simulink library "lib_LargeBuildingModel"  (R2026a)
settings: Solver=VariableStepAuto
libraries: WallSelector_lib x380, ExternalWall_lib x188, RoomWithAirVolume x140, fl_lib x139, RoomLevelControl_lib x1
(part 6 of 12)

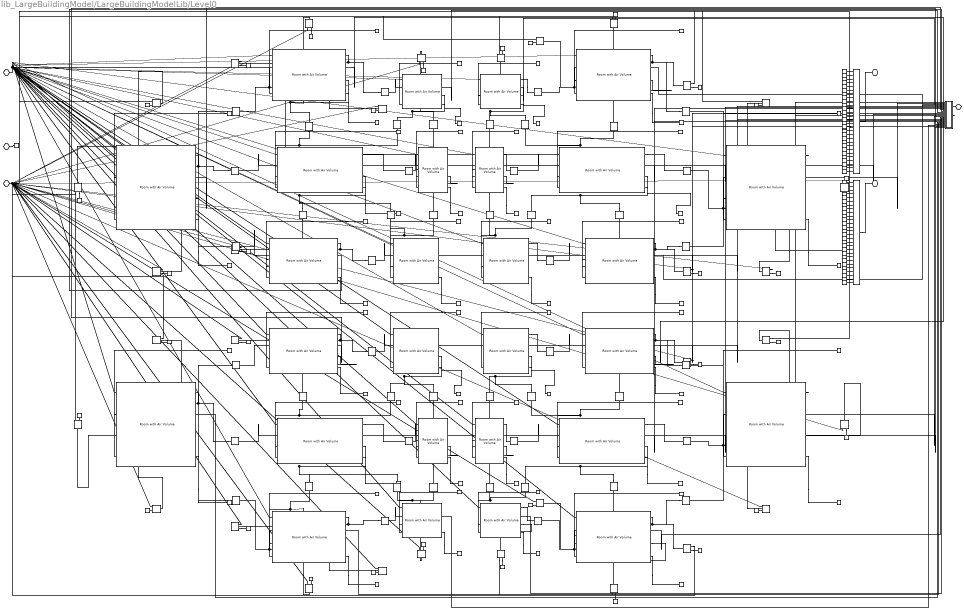
== system lib_LargeBuildingModel/LargeBuildingModelLib/Level0 ==
  note: A1R1 (LivingRoom_A)
  note: A1R2 (Bedroom_A)
  note: A1R3 (Kitchen_A)
  note: A1R4 (Bathroom_A)
  note: A1R5 (FireExit_A)
  note: A1R6 (Lobby1_A)
  note: A1R7 (Lobby2_A)
  note: A2R1 (LivingRoom_B)
  note: A2R2 (Bedroom_B)
  note: A2R3 (Kitchen_B)
  note: A2R4 (Bathroom_B)
  note: A2R5 (FireExit_B)
  note: A2R6 (Lobby1_B)
  note: A2R7 (Lobby2_B)
  note: A3R1 (LivingRoom_C)
  note: A3R2 (Bedroom_C)
  note: A3R3 (Kitchen_C)
  note: A3R4 (Bathroom_C)
  note: A3R5 (FireExit_C)
  note: A3R6 (Lobby1_C)
  note: A3R7 (Lobby2_C)
  note: A4R1 (LivingRoom_D)
  note: A4R2 (Bedroom_D)
  note: A4R3 (Kitchen_D)
  note: A4R4 (Bathroom_D)
  note: A4R5 (FireExit_D)
  note: A4R6 (Lobby1_D)
  note: A4R7 (Lobby2_D)
  Amb{1..32} (32 alike) : ConnectionLabel  Label=A
  AmbPort : ConnectionLabel  Label=A
  ArrayBottom : SimscapeArrayConnection  Domain=foundation.thermal.thermal  ConcatenateDimension=1  NumScalarElements=28
  ArrayTop : SimscapeArrayConnection  Domain=foundation.thermal.thermal  ConcatenateDimension=1  NumScalarElements=28
  Bottom1 : ConnectionLabel  Label=Bottom1
  Bottom10 : ConnectionLabel  Label=Bottom10
  Bottom10Lib : ConnectionLabel  Label=Bottom10
  Bottom11 : ConnectionLabel  Label=Bottom11
  Bottom11Lib : ConnectionLabel  Label=Bottom11
  Bottom12 : ConnectionLabel  Label=Bottom12
  Bottom12Lib : ConnectionLabel  Label=Bottom12
  Bottom13 : ConnectionLabel  Label=Bottom13
  Bottom13Lib : ConnectionLabel  Label=Bottom13
  Bottom14 : ConnectionLabel  Label=Bottom14
  Bottom14Lib : ConnectionLabel  Label=Bottom14
  Bottom15 : ConnectionLabel  Label=Bottom15
  Bottom15Lib : ConnectionLabel  Label=Bottom15
  Bottom16 : ConnectionLabel  Label=Bottom16
  Bottom16Lib : ConnectionLabel  Label=Bottom16
  Bottom17 : ConnectionLabel  Label=Bottom17
  Bottom17Lib : ConnectionLabel  Label=Bottom17
  Bottom18 : ConnectionLabel  Label=Bottom18
  Bottom18Lib : ConnectionLabel  Label=Bottom18
  Bottom19 : ConnectionLabel  Label=Bottom19
  Bottom19Lib : ConnectionLabel  Label=Bottom19
  Bottom1Lib : ConnectionLabel  Label=Bottom1
  Bottom2 : ConnectionLabel  Label=Bottom2
  Bottom20 : ConnectionLabel  Label=Bottom20
  Bottom20Lib : ConnectionLabel  Label=Bottom20
  Bottom21 : ConnectionLabel  Label=Bottom21
  Bottom21Lib : ConnectionLabel  Label=Bottom21
  Bottom22 : ConnectionLabel  Label=Bottom22
  Bottom22Lib : ConnectionLabel  Label=Bottom22
  Bottom23 : ConnectionLabel  Label=Bottom23
  Bottom23Lib : ConnectionLabel  Label=Bottom23
  Bottom24 : ConnectionLabel  Label=Bottom24
  Bottom24Lib : ConnectionLabel  Label=Bottom24
  Bottom25 : ConnectionLabel  Label=Bottom25
  Bottom25Lib : ConnectionLabel  Label=Bottom25
  Bottom26 : ConnectionLabel  Label=Bottom26
  Bottom26Lib : ConnectionLabel  Label=Bottom26
  Bottom27 : ConnectionLabel  Label=Bottom27
  Bottom27Lib : ConnectionLabel  Label=Bottom27
  Bottom28 : ConnectionLabel  Label=Bottom28
  Bottom28Lib : ConnectionLabel  Label=Bottom28
  Bottom2Lib : ConnectionLabel  Label=Bottom2
  Bottom3 : ConnectionLabel  Label=Bottom3
  Bottom3Lib : ConnectionLabel  Label=Bottom3
  Bottom4 : ConnectionLabel  Label=Bottom4
  Bottom4Lib : ConnectionLabel  Label=Bottom4
  Bottom5 : ConnectionLabel  Label=Bottom5
  Bottom5Lib : ConnectionLabel  Label=Bottom5
  Bottom6 : ConnectionLabel  Label=Bottom6
  Bottom6Lib : ConnectionLabel  Label=Bottom6
  Bottom7 : ConnectionLabel  Label=Bottom7
  Bottom7Lib : ConnectionLabel  Label=Bottom7
  Bottom8 : ConnectionLabel  Label=Bottom8
  Bottom8Lib : ConnectionLabel  Label=Bottom8
  Bottom9 : ConnectionLabel  Label=Bottom9
  Bottom9Lib : ConnectionLabel  Label=Bottom9
  ExtWall (A1R2W1) : ExternalWall_lib/Wall External  extWallModel=wallExternalModelOption.wallSolarWin  wallLength=4.2672 % Parameterized on : 13-Jun-2026 10:47:11 m  wallHeight=3.048 % Parameterized on : 13-Jun-2026 10:47:11 m  wallThickness=0.07 % Parameterized on : 13-Jun-2026 10:47:11 m  wallMaterialDen=2000 % Parameterized on : 13-Jun-2026 10:47:16 kg/m^3  wallMaterialCp=1100 % Parameterized on : 13-Jun-2026 10:47:16 J/(K*kg)  wallAbsorptivity=0.6 % Parameterized on : 13-Jun-2026 10:47:16  wallThermalK=1.4 % Parameterized on : 13-Jun-2026 10:47:16 W/(K*m)  winLength=3.0174 % Parameterized on : 13-Jun-2026 10:47:11 m  winHeight=2.1553 % Parameterized on : 13-Jun-2026 10:47:11 m  winThickness=0.005 % Parameterized on : 13-Jun-2026 10:47:16 m  winMaterialDen=4000 % Parameterized on : 13-Jun-2026 10:47:17 kg/m^3  winMaterialCp=840 % Parameterized on : 13-Jun-2026 10:47:17 J/(K*kg)  winAbsorptivity=0.4 % Parameterized on : 13-Jun-2026 10:47:17  winThermalK=1 % Parameterized on : 13-Jun-2026 10:47:17 W/(K*m)  winTransmissivity=0.2 % Parameterized on : 13-Jun-2026 10:47:17  ventLength=0.1 m  ventHeight=0.1 m  extToWallHTC=20 % Parameterized on : 13-Jun-2026 10:47:16 W/(K*m^2)  intToRoomHTC=30 % Parameterized on : 13-Jun-2026 10:47:16 W/(K*m^2)  iniT=300 % Parameterized on : 13-Jun-2026 10:47:16 K  latitude=5  longitude=5  localTime=5  dayLightS=0  surfAngle=90 % Parameterized on : 13-Jun-2026 10:47:11 deg  surfUnitV=[0 -1] % Parameterized on : 13-Jun-2026 10:47:11  startYear=2025  startMonth=1  startDay=1  startHr=1  numHrsData=24  interp_method=simscape.enum.interpolation.linear  extrap_method=simscape.enum.extrapolation.nearest
  ExtWall (A1R2W3) : ExternalWall_lib/Wall External  extWallModel=wallExternalModelOption.wallSolarWin  wallLength=4.2672 % Parameterized on : 13-Jun-2026 10:47:11 m  wallHeight=3.048 % Parameterized on : 13-Jun-2026 10:47:11 m  wallThickness=0.07 % Parameterized on : 13-Jun-2026 10:47:11 m  wallMaterialDen=2000 % Parameterized on : 13-Jun-2026 10:47:17 kg/m^3  wallMaterialCp=1100 % Parameterized on : 13-Jun-2026 10:47:17 J/(K*kg)  wallAbsorptivity=0.6 % Parameterized on : 13-Jun-2026 10:47:17  wallThermalK=1.4 % Parameterized on : 13-Jun-2026 10:47:17 W/(K*m)  winLength=3.3054 % Parameterized on : 13-Jun-2026 10:47:12 m  winHeight=2.361 % Parameterized on : 13-Jun-2026 10:47:12 m  winThickness=0.005 % Parameterized on : 13-Jun-2026 10:47:17 m  winMaterialDen=4000 % Parameterized on : 13-Jun-2026 10:47:17 kg/m^3  winMaterialCp=840 % Parameterized on : 13-Jun-2026 10:47:17 J/(K*kg)  winAbsorptivity=0.4 % Parameterized on : 13-Jun-2026 10:47:17  winThermalK=1 % Parameterized on : 13-Jun-2026 10:47:17 W/(K*m)  winTransmissivity=0.2 % Parameterized on : 13-Jun-2026 10:47:17  ventLength=0.1 m  ventHeight=0.1 m  extToWallHTC=20 % Parameterized on : 13-Jun-2026 10:47:17 W/(K*m^2)  intToRoomHTC=30 % Parameterized on : 13-Jun-2026 10:47:17 W/(K*m^2)  iniT=300 % Parameterized on : 13-Jun-2026 10:47:17 K  latitude=5  longitude=5  localTime=5  dayLightS=0  surfAngle=90 % Parameterized on : 13-Jun-2026 10:47:11 deg  surfUnitV="[0  1] % Parameterized on : 13-Jun-2026 10:47:11"  startYear=2025  startMonth=1  startDay=1  startHr=1  numHrsData=24  interp_method=simscape.enum.interpolation.linear  extrap_method=simscape.enum.extrapolation.nearest
  ExtWall (A1R2W4) : ExternalWall_lib/Wall External  extWallModel=wallExternalModelOption.wallSolar  wallLength=4.572 % Parameterized on : 13-Jun-2026 10:47:12 m  wallHeight=3.048 % Parameterized on : 13-Jun-2026 10:47:12 m  wallThickness=0.07 % Parameterized on : 13-Jun-2026 10:47:12 m  wallMaterialDen=2000 % Parameterized on : 13-Jun-2026 10:47:17 kg/m^3  wallMaterialCp=1100 % Parameterized on : 13-Jun-2026 10:47:17 J/(K*kg)  wallAbsorptivity=0.6 % Parameterized on : 13-Jun-2026 10:47:17  wallThermalK=1.4 % Parameterized on : 13-Jun-2026 10:47:17 W/(K*m)  winLength=1 m  winHeight=0.5 m  winThickness=0.007 m  winMaterialDen=2500 kg/m^3  winMaterialCp=787 J/(K*kg)  winAbsorptivity=0.35  winThermalK=1 W/(K*m)  winTransmissivity=0.45  ventLength=0.1 m  ventHeight=0.1 m  extToWallHTC=20 % Parameterized on : 13-Jun-2026 10:47:17 W/(K*m^2)  intToRoomHTC=30 % Parameterized on : 13-Jun-2026 10:47:17 W/(K*m^2)  iniT=300 % Parameterized on : 13-Jun-2026 10:47:17 K  latitude=5  longitude=5  localTime=5  dayLightS=0  surfAngle=90 % Parameterized on : 13-Jun-2026 10:47:12 deg  surfUnitV="[1  0] % Parameterized on : 13-Jun-2026 10:47:12"  startYear=2025  startMonth=1  startDay=1  startHr=1  numHrsData=24  interp_method=simscape.enum.interpolation.linear  extrap_method=simscape.enum.extrapolation.nearest
  ExtWall (A1R3W1) : ExternalWall_lib/Wall External  extWallModel=wallExternalModelOption.wallSolarWin  wallLength=2.7432 % Parameterized on : 13-Jun-2026 10:47:12 m  wallHeight=3.048 % Parameterized on : 13-Jun-2026 10:47:12 m  wallThickness=0.07 % Parameterized on : 13-Jun-2026 10:47:12 m  wallMaterialDen=2000 % Parameterized on : 13-Jun-2026 10:47:17 kg/m^3  wallMaterialCp=1100 % Parameterized on : 13-Jun-2026 10:47:17 J/(K*kg)  wallAbsorptivity=0.6 % Parameterized on : 13-Jun-2026 10:47:17  wallThermalK=1.4 % Parameterized on : 13-Jun-2026 10:47:17 W/(K*m)  winLength=2.4536 % Parameterized on : 13-Jun-2026 10:47:12 m  winHeight=2.7262 % Parameterized on : 13-Jun-2026 10:47:12 m  winThickness=0.005 % Parameterized on : 13-Jun-2026 10:47:17 m  winMaterialDen=4000 % Parameterized on : 13-Jun-2026 10:47:17 kg/m^3  winMaterialCp=840 % Parameterized on : 13-Jun-2026 10:47:17 J/(K*kg)  winAbsorptivity=0.4 % Parameterized on : 13-Jun-2026 10:47:17  winThermalK=1 % Parameterized on : 13-Jun-2026 10:47:17 W/(K*m)  winTransmissivity=0.2 % Parameterized on : 13-Jun-2026 10:47:17  ventLength=0.1 m  ventHeight=0.1 m  extToWallHTC=20 % Parameterized on : 13-Jun-2026 10:47:17 W/(K*m^2)  intToRoomHTC=30 % Parameterized on : 13-Jun-2026 10:47:17 W/(K*m^2)  iniT=300 % Parameterized on : 13-Jun-2026 10:47:17 K  latitude=5  longitude=5  localTime=5  dayLightS=0  surfAngle=90 % Parameterized on : 13-Jun-2026 10:47:12 deg  surfUnitV="[-1  0] % Parameterized on : 13-Jun-2026 10:47:12"  startYear=2025  startMonth=1  startDay=1  startHr=1  numHrsData=24  interp_method=simscape.enum.interpolation.linear  extrap_method=simscape.enum.extrapolation.nearest
  ExtWall (A1R3W3) : ExternalWall_lib/Wall External  extWallModel=wallExternalModelOption.wallSolarWin  wallLength=2.7432 % Parameterized on : 13-Jun-2026 10:47:12 m  wallHeight=3.048 % Parameterized on : 13-Jun-2026 10:47:12 m  wallThickness=0.07 % Parameterized on : 13-Jun-2026 10:47:12 m  wallMaterialDen=2000 % Parameterized on : 13-Jun-2026 10:47:17 kg/m^3  wallMaterialCp=1100 % Parameterized on : 13-Jun-2026 10:47:17 J/(K*kg)  wallAbsorptivity=0.6 % Parameterized on : 13-Jun-2026 10:47:17  wallThermalK=1.4 % Parameterized on : 13-Jun-2026 10:47:17 W/(K*m)  winLength=1.9397 % Parameterized on : 13-Jun-2026 10:47:12 m  winHeight=2.1553 % Parameterized on : 13-Jun-2026 10:47:12 m  winThickness=0.005 % Parameterized on : 13-Jun-2026 10:47:17 m  winMaterialDen=4000 % Parameterized on : 13-Jun-2026 10:47:17 kg/m^3  winMaterialCp=840 % Parameterized on : 13-Jun-2026 10:47:17 J/(K*kg)  winAbsorptivity=0.4 % Parameterized on : 13-Jun-2026 10:47:17  winThermalK=1 % Parameterized on : 13-Jun-2026 10:47:17 W/(K*m)  winTransmissivity=0.2 % Parameterized on : 13-Jun-2026 10:47:17  ventLength=0.1 m  ventHeight=0.1 m  extToWallHTC=20 % Parameterized on : 13-Jun-2026 10:47:17 W/(K*m^2)  intToRoomHTC=30 % Parameterized on : 13-Jun-2026 10:47:17 W/(K*m^2)  iniT=300 % Parameterized on : 13-Jun-2026 10:47:17 K  latitude=5  longitude=5  localTime=5  dayLightS=0  surfAngle=90 % Parameterized on : 13-Jun-2026 10:47:12 deg  surfUnitV="[1  0] % Parameterized on : 13-Jun-2026 10:47:12"  startYear=2025  startMonth=1  startDay=1  startHr=1  numHrsData=24  interp_method=simscape.enum.interpolation.linear  extrap_method=simscape.enum.extrapolation.nearest
  ExtWall (A1R3W4) : ExternalWall_lib/Wall External  extWallModel=wallExternalModelOption.wallSolar  wallLength=3.9624 % Parameterized on : 13-Jun-2026 10:47:12 m  wallHeight=3.048 % Parameterized on : 13-Jun-2026 10:47:12 m  wallThickness=0.07 % Parameterized on : 13-Jun-2026 10:47:12 m  wallMaterialDen=2000 % Parameterized on : 13-Jun-2026 10:47:17 kg/m^3  wallMaterialCp=1100 % Parameterized on : 13-Jun-2026 10:47:17 J/(K*kg)  wallAbsorptivity=0.6 % Parameterized on : 13-Jun-2026 10:47:17  wallThermalK=1.4 % Parameterized on : 13-Jun-2026 10:47:17 W/(K*m)  winLength=1 m  winHeight=0.5 m  winThickness=0.007 m  winMaterialDen=2500 kg/m^3  winMaterialCp=787 J/(K*kg)  winAbsorptivity=0.35  winThermalK=1 W/(K*m)  winTransmissivity=0.45  ventLength=0.1 m  ventHeight=0.1 m  extToWallHTC=20 % Parameterized on : 13-Jun-2026 10:47:17 W/(K*m^2)  intToRoomHTC=30 % Parameterized on : 13-Jun-2026 10:47:17 W/(K*m^2)  iniT=300 % Parameterized on : 13-Jun-2026 10:47:17 K  latitude=5  longitude=5  localTime=5  dayLightS=0  surfAngle=90 % Parameterized on : 13-Jun-2026 10:47:12 deg  surfUnitV=[0 -1] % Parameterized on : 13-Jun-2026 10:47:12  startYear=2025  startMonth=1  startDay=1  startHr=1  numHrsData=24  interp_method=simscape.enum.interpolation.linear  extrap_method=simscape.enum.extrapolation.nearest
  ExtWall (A1R4W3) : ExternalWall_lib/Wall External  extWallModel=wallExternalModelOption.wallSolar  wallLength=2.4384 % Parameterized on : 13-Jun-2026 10:47:12 m  wallHeight=3.048 % Parameterized on : 13-Jun-2026 10:47:12 m  wallThickness=0.07 % Parameterized on : 13-Jun-2026 10:47:12 m  wallMaterialDen=2000 % Parameterized on : 13-Jun-2026 10:47:17 kg/m^3  wallMaterialCp=1100 % Parameterized on : 13-Jun-2026 10:47:17 J/(K*kg)  wallAbsorptivity=0.6 % Parameterized on : 13-Jun-2026 10:47:17  wallThermalK=1.4 % Parameterized on : 13-Jun-2026 10:47:17 W/(K*m)  winLength=1 m  winHeight=0.5 m  winThickness=0.007 m  winMaterialDen=2500 kg/m^3  winMaterialCp=787 J/(K*kg)  winAbsorptivity=0.35  winThermalK=1 W/(K*m)  winTransmissivity=0.45  ventLength=0.1 m  ventHeight=0.1 m  extToWallHTC=20 % Parameterized on : 13-Jun-2026 10:47:17 W/(K*m^2)  intToRoomHTC=30 % Parameterized on : 13-Jun-2026 10:47:17 W/(K*m^2)  iniT=300 % Parameterized on : 13-Jun-2026 10:47:17 K  latitude=5  longitude=5  localTime=5  dayLightS=0  surfAngle=90 % Parameterized on : 13-Jun-2026 10:47:12 deg  surfUnitV="[1  0] % Parameterized on : 13-Jun-2026 10:47:12"  startYear=2025  startMonth=1  startDay=1  startHr=1  numHrsData=24  interp_method=simscape.enum.interpolation.linear  extrap_method=simscape.enum.extrapolation.nearest
  ExtWall (A1R5W4) : ExternalWall_lib/Wall External  extWallModel=wallExternalModelOption.wallSolar  wallLength=2.1336 % Parameterized on : 13-Jun-2026 10:47:12 m  wallHeight=3.048 % Parameterized on : 13-Jun-2026 10:47:12 m  wallThickness=0.07 % Parameterized on : 13-Jun-2026 10:47:12 m  wallMaterialDen=2000 % Parameterized on : 13-Jun-2026 10:47:17 kg/m^3  wallMaterialCp=1100 % Parameterized on : 13-Jun-2026 10:47:17 J/(K*kg)  wallAbsorptivity=0.6 % Parameterized on : 13-Jun-2026 10:47:17  wallThermalK=1.4 % Parameterized on : 13-Jun-2026 10:47:17 W/(K*m)  winLength=1 m  winHeight=0.5 m  winThickness=0.007 m  winMaterialDen=2500 kg/m^3  winMaterialCp=787 J/(K*kg)  winAbsorptivity=0.35  winThermalK=1 W/(K*m)  winTransmissivity=0.45  ventLength=0.1 m  ventHeight=0.1 m  extToWallHTC=20 % Parameterized on : 13-Jun-2026 10:47:17 W/(K*m^2)  intToRoomHTC=30 % Parameterized on : 13-Jun-2026 10:47:17 W/(K*m^2)  iniT=300 % Parameterized on : 13-Jun-2026 10:47:17 K  latitude=5  longitude=5  localTime=5  dayLightS=0  surfAngle=90 % Parameterized on : 13-Jun-2026 10:47:12 deg  surfUnitV="[-6.0708e-17          -1] % Parameterized on : 13-Jun-2026 10:47:12"  startYear=2025  startMonth=1  startDay=1  startHr=1  numHrsData=24  interp_method=simscape.enum.interpolation.linear  extrap_method=simscape.enum.extrapolation.nearest
  ExtWall (A2R2W1) : ExternalWall_lib/Wall External  extWallModel=wallExternalModelOption.wallSolarWin  wallLength=4.2672 % Parameterized on : 13-Jun-2026 10:47:12 m  wallHeight=3.048 % Parameterized on : 13-Jun-2026 10:47:12 m  wallThickness=0.07 % Parameterized on : 13-Jun-2026 10:47:12 m  wallMaterialDen=2000 % Parameterized on : 13-Jun-2026 10:47:17 kg/m^3  wallMaterialCp=1100 % Parameterized on : 13-Jun-2026 10:47:17 J/(K*kg)  wallAbsorptivity=0.6 % Parameterized on : 13-Jun-2026 10:47:17  wallThermalK=1.4 % Parameterized on : 13-Jun-2026 10:47:17 W/(K*m)  winLength=3.3054 % Parameterized on : 13-Jun-2026 10:47:12 m  winHeight=2.361 % Parameterized on : 13-Jun-2026 10:47:12 m  winThickness=0.005 % Parameterized on : 13-Jun-2026 10:47:17 m  winMaterialDen=4000 % Parameterized on : 13-Jun-2026 10:47:17 kg/m^3  winMaterialCp=840 % Parameterized on : 13-Jun-2026 10:47:17 J/(K*kg)  winAbsorptivity=0.4 % Parameterized on : 13-Jun-2026 10:47:17  winThermalK=1 % Parameterized on : 13-Jun-2026 10:47:17 W/(K*m)  winTransmissivity=0.2 % Parameterized on : 13-Jun-2026 10:47:17  ventLength=0.1 m  ventHeight=0.1 m  extToWallHTC=20 % Parameterized on : 13-Jun-2026 10:47:17 W/(K*m^2)  intToRoomHTC=30 % Parameterized on : 13-Jun-2026 10:47:17 W/(K*m^2)  iniT=300 % Parameterized on : 13-Jun-2026 10:47:17 K  latitude=5  longitude=5  localTime=5  dayLightS=0  surfAngle=90 % Parameterized on : 13-Jun-2026 10:47:12 deg  surfUnitV=[0 -1] % Parameterized on : 13-Jun-2026 10:47:12  startYear=2025  startMonth=1  startDay=1  startHr=1  numHrsData=24  interp_method=simscape.enum.interpolation.linear  extrap_method=simscape.enum.extrapolation.nearest
  ExtWall (A2R2W2) : ExternalWall_lib/Wall External  extWallModel=wallExternalModelOption.wallSolar  wallLength=4.572 % Parameterized on : 13-Jun-2026 10:47:12 m  wallHeight=3.048 % Parameterized on : 13-Jun-2026 10:47:12 m  wallThickness=0.07 % Parameterized on : 13-Jun-2026 10:47:12 m  wallMaterialDen=2000 % Parameterized on : 13-Jun-2026 10:47:17 kg/m^3  wallMaterialCp=1100 % Parameterized on : 13-Jun-2026 10:47:17 J/(K*kg)  wallAbsorptivity=0.6 % Parameterized on : 13-Jun-2026 10:47:17  wallThermalK=1.4 % Parameterized on : 13-Jun-2026 10:47:17 W/(K*m)  winLength=1 m  winHeight=0.5 m  winThickness=0.007 m  winMaterialDen=2500 kg/m^3  winMaterialCp=787 J/(K*kg)  winAbsorptivity=0.35  winThermalK=1 W/(K*m)  winTransmissivity=0.45  ventLength=0.1 m  ventHeight=0.1 m  extToWallHTC=20 % Parameterized on : 13-Jun-2026 10:47:17 W/(K*m^2)  intToRoomHTC=30 % Parameterized on : 13-Jun-2026 10:47:17 W/(K*m^2)  iniT=300 % Parameterized on : 13-Jun-2026 10:47:17 K  latitude=5  longitude=5  localTime=5  dayLightS=0  surfAngle=90 % Parameterized on : 13-Jun-2026 10:47:12 deg  surfUnitV="[-1  0] % Parameterized on : 13-Jun-2026 10:47:12"  startYear=2025  startMonth=1  startDay=1  startHr=1  numHrsData=24  interp_method=simscape.enum.interpolation.linear  extrap_method=simscape.enum.extrapolation.nearest
  ExtWall (A2R2W3) : ExternalWall_lib/Wall External  extWallModel=wallExternalModelOption.wallSolarWin  wallLength=4.2672 % Parameterized on : 13-Jun-2026 10:47:12 m  wallHeight=3.048 % Parameterized on : 13-Jun-2026 10:47:12 m  wallThickness=0.07 % Parameterized on : 13-Jun-2026 10:47:12 m  wallMaterialDen=2000 % Parameterized on : 13-Jun-2026 10:47:17 kg/m^3  wallMaterialCp=1100 % Parameterized on : 13-Jun-2026 10:47:17 J/(K*kg)  wallAbsorptivity=0.6 % Parameterized on : 13-Jun-2026 10:47:17  wallThermalK=1.4 % Parameterized on : 13-Jun-2026 10:47:17 W/(K*m)  winLength=3.8167 % Parameterized on : 13-Jun-2026 10:47:12 m  winHeight=2.7262 % Parameterized on : 13-Jun-2026 10:47:12 m  winThickness=0.005 % Parameterized on : 13-Jun-2026 10:47:17 m  winMaterialDen=4000 % Parameterized on : 13-Jun-2026 10:47:17 kg/m^3  winMaterialCp=840 % Parameterized on : 13-Jun-2026 10:47:17 J/(K*kg)  winAbsorptivity=0.4 % Parameterized on : 13-Jun-2026 10:47:17  winThermalK=1 % Parameterized on : 13-Jun-2026 10:47:17 W/(K*m)  winTransmissivity=0.2 % Parameterized on : 13-Jun-2026 10:47:17  ventLength=0.1 m  ventHeight=0.1 m  extToWallHTC=20 % Parameterized on : 13-Jun-2026 10:47:17 W/(K*m^2)  intToRoomHTC=30 % Parameterized on : 13-Jun-2026 10:47:17 W/(K*m^2)  iniT=300 % Parameterized on : 13-Jun-2026 10:47:17 K  latitude=5  longitude=5  localTime=5  dayLightS=0  surfAngle=90 % Parameterized on : 13-Jun-2026 10:47:12 deg  surfUnitV="[0  1] % Parameterized on : 13-Jun-2026 10:47:12"  startYear=2025  startMonth=1  startDay=1  startHr=1  numHrsData=24  interp_method=simscape.enum.interpolation.linear  extrap_method=simscape.enum.extrapolation.nearest
  ExtWall (A2R3W1) : ExternalWall_lib/Wall External  extWallModel=wallExternalModelOption.wallSolarWin  wallLength=2.7432 % Parameterized on : 13-Jun-2026 10:47:12 m  wallHeight=3.048 % Parameterized on : 13-Jun-2026 10:47:12 m  wallThickness=0.07 % Parameterized on : 13-Jun-2026 10:47:12 m  wallMaterialDen=2000 % Parameterized on : 13-Jun-2026 10:47:17 kg/m^3  wallMaterialCp=1100 % Parameterized on : 13-Jun-2026 10:47:17 J/(K*kg)  wallAbsorptivity=0.6 % Parameterized on : 13-Jun-2026 10:47:17  wallThermalK=1.4 % Parameterized on : 13-Jun-2026 10:47:17 W/(K*m)  winLength=1.9397 % Parameterized on : 13-Jun-2026 10:47:12 m  winHeight=2.1553 % Parameterized on : 13-Jun-2026 10:47:12 m  winThickness=0.005 % Parameterized on : 13-Jun-2026 10:47:17 m  winMaterialDen=4000 % Parameterized on : 13-Jun-2026 10:47:17 kg/m^3  winMaterialCp=840 % Parameterized on : 13-Jun-2026 10:47:17 J/(K*kg)  winAbsorptivity=0.4 % Parameterized on : 13-Jun-2026 10:47:17  winThermalK=1 % Parameterized on : 13-Jun-2026 10:47:17 W/(K*m)  winTransmissivity=0.2 % Parameterized on : 13-Jun-2026 10:47:17  ventLength=0.1 m  ventHeight=0.1 m  extToWallHTC=20 % Parameterized on : 13-Jun-2026 10:47:17 W/(K*m^2)  intToRoomHTC=30 % Parameterized on : 13-Jun-2026 10:47:17 W/(K*m^2)  iniT=300 % Parameterized on : 13-Jun-2026 10:47:17 K  latitude=5  longitude=5  localTime=5  dayLightS=0  surfAngle=90 % Parameterized on : 13-Jun-2026 10:47:12 deg  surfUnitV="[1  0] % Parameterized on : 13-Jun-2026 10:47:12"  startYear=2025  startMonth=1  startDay=1  startHr=1  numHrsData=24  interp_method=simscape.enum.interpolation.linear  extrap_method=simscape.enum.extrapolation.nearest
  ExtWall (A2R3W2) : ExternalWall_lib/Wall External  extWallModel=wallExternalModelOption.wallSolarWin  wallLength=3.9624 % Parameterized on : 13-Jun-2026 10:47:12 m  wallHeight=3.048 % Parameterized on : 13-Jun-2026 10:47:12 m  wallThickness=0.07 % Parameterized on : 13-Jun-2026 10:47:12 m  wallMaterialDen=2000 % Parameterized on : 13-Jun-2026 10:47:17 kg/m^3  wallMaterialCp=1100 % Parameterized on : 13-Jun-2026 10:47:17 J/(K*kg)  wallAbsorptivity=0.6 % Parameterized on : 13-Jun-2026 10:47:17  wallThermalK=1.4 % Parameterized on : 13-Jun-2026 10:47:17 W/(K*m)  winLength=2.8018 % Parameterized on : 13-Jun-2026 10:47:12 m  winHeight=2.1553 % Parameterized on : 13-Jun-2026 10:47:12 m  winThickness=0.005 % Parameterized on : 13-Jun-2026 10:47:17 m  winMaterialDen=4000 % Parameterized on : 13-Jun-2026 10:47:17 kg/m^3  winMaterialCp=840 % Parameterized on : 13-Jun-2026 10:47:17 J/(K*kg)  winAbsorptivity=0.4 % Parameterized on : 13-Jun-2026 10:47:17  winThermalK=1 % Parameterized on : 13-Jun-2026 10:47:17 W/(K*m)  winTransmissivity=0.2 % Parameterized on : 13-Jun-2026 10:47:17  ventLength=0.1 m  ventHeight=0.1 m  extToWallHTC=20 % Parameterized on : 13-Jun-2026 10:47:17 W/(K*m^2)  intToRoomHTC=30 % Parameterized on : 13-Jun-2026 10:47:17 W/(K*m^2)  iniT=300 % Parameterized on : 13-Jun-2026 10:47:17 K  latitude=5  longitude=5  localTime=5  dayLightS=0  surfAngle=90 % Parameterized on : 13-Jun-2026 10:47:12 deg  surfUnitV=[0 -1] % Parameterized on : 13-Jun-2026 10:47:12  startYear=2025  startMonth=1  startDay=1  startHr=1  numHrsData=24  interp_method=simscape.enum.interpolation.linear  extrap_method=simscape.enum.extrapolation.nearest
  ExtWall (A2R3W3) : ExternalWall_lib/Wall External  extWallModel=wallExternalModelOption.wallSolar  wallLength=2.7432 % Parameterized on : 13-Jun-2026 10:47:12 m  wallHeight=3.048 % Parameterized on : 13-Jun-2026 10:47:12 m  wallThickness=0.07 % Parameterized on : 13-Jun-2026 10:47:12 m  wallMaterialDen=2000 % Parameterized on : 13-Jun-2026 10:47:17 kg/m^3  wallMaterialCp=1100 % Parameterized on : 13-Jun-2026 10:47:17 J/(K*kg)  wallAbsorptivity=0.6 % Parameterized on : 13-Jun-2026 10:47:17  wallThermalK=1.4 % Parameterized on : 13-Jun-2026 10:47:17 W/(K*m)  winLength=1 m  winHeight=0.5 m  winThickness=0.007 m  winMaterialDen=2500 kg/m^3  winMaterialCp=787 J/(K*kg)  winAbsorptivity=0.35  winThermalK=1 W/(K*m)  winTransmissivity=0.45  ventLength=0.1 m  ventHeight=0.1 m  extToWallHTC=20 % Parameterized on : 13-Jun-2026 10:47:17 W/(K*m^2)  intToRoomHTC=30 % Parameterized on : 13-Jun-2026 10:47:17 W/(K*m^2)  iniT=300 % Parameterized on : 13-Jun-2026 10:47:17 K  latitude=5  longitude=5  localTime=5  dayLightS=0  surfAngle=90 % Parameterized on : 13-Jun-2026 10:47:12 deg  surfUnitV="[-1  0] % Parameterized on : 13-Jun-2026 10:47:12"  startYear=2025  startMonth=1  startDay=1  startHr=1  numHrsData=24  interp_method=simscape.enum.interpolation.linear  extrap_method=simscape.enum.extrapolation.nearest
  ExtWall (A2R4W3) : ExternalWall_lib/Wall External  extWallModel=wallExternalModelOption.wallSolar  wallLength=2.4384 % Parameterized on : 13-Jun-2026 10:47:12 m  wallHeight=3.048 % Parameterized on : 13-Jun-2026 10:47:12 m  wallThickness=0.07 % Parameterized on : 13-Jun-2026 10:47:12 m  wallMaterialDen=2000 % Parameterized on : 13-Jun-2026 10:47:17 kg/m^3  wallMaterialCp=1100 % Parameterized on : 13-Jun-2026 10:47:17 J/(K*kg)  wallAbsorptivity=0.6 % Parameterized on : 13-Jun-2026 10:47:17  wallThermalK=1.4 % Parameterized on : 13-Jun-2026 10:47:17 W/(K*m)  winLength=1 m  winHeight=0.5 m  winThickness=0.007 m  winMaterialDen=2500 kg/m^3  winMaterialCp=787 J/(K*kg)  winAbsorptivity=0.35  winThermalK=1 W/(K*m)  winTransmissivity=0.45  ventLength=0.1 m  ventHeight=0.1 m  extToWallHTC=20 % Parameterized on : 13-Jun-2026 10:47:17 W/(K*m^2)  intToRoomHTC=30 % Parameterized on : 13-Jun-2026 10:47:17 W/(K*m^2)  iniT=300 % Parameterized on : 13-Jun-2026 10:47:17 K  latitude=5  longitude=5  localTime=5  dayLightS=0  surfAngle=90 % Parameterized on : 13-Jun-2026 10:47:12 deg  surfUnitV="[-1  0] % Parameterized on : 13-Jun-2026 10:47:12"  startYear=2025  startMonth=1  startDay=1  startHr=1  numHrsData=24  interp_method=simscape.enum.interpolation.linear  extrap_method=simscape.enum.extrapolation.nearest
  ExtWall (A2R5W2) : ExternalWall_lib/Wall External  extWallModel=wallExternalModelOption.wallSolar  wallLength=2.1336 % Parameterized on : 13-Jun-2026 10:47:12 m  wallHeight=3.048 % Parameterized on : 13-Jun-2026 10:47:12 m  wallThickness=0.07 % Parameterized on : 13-Jun-2026 10:47:12 m  wallMaterialDen=2000 % Parameterized on : 13-Jun-2026 10:47:17 kg/m^3  wallMaterialCp=1100 % Parameterized on : 13-Jun-2026 10:47:17 J/(K*kg)  wallAbsorptivity=0.6 % Parameterized on : 13-Jun-2026 10:47:17  wallThermalK=1.4 % Parameterized on : 13-Jun-2026 10:47:17 W/(K*m)  winLength=1 m  winHeight=0.5 m  winThickness=0.007 m  winMaterialDen=2500 kg/m^3  winMaterialCp=787 J/(K*kg)  winAbsorptivity=0.35  winThermalK=1 W/(K*m)  winTransmissivity=0.45  ventLength=0.1 m  ventHeight=0.1 m  extToWallHTC=20 % Parameterized on : 13-Jun-2026 10:47:17 W/(K*m^2)  intToRoomHTC=30 % Parameterized on : 13-Jun-2026 10:47:17 W/(K*m^2)  iniT=300 % Parameterized on : 13-Jun-2026 10:47:17 K  latitude=5  longitude=5  localTime=5  dayLightS=0  surfAngle=90 % Parameterized on : 13-Jun-2026 10:47:12 deg  surfUnitV=[0 -1] % Parameterized on : 13-Jun-2026 10:47:12  startYear=2025  startMonth=1  startDay=1  startHr=1  numHrsData=24  interp_method=simscape.enum.interpolation.linear  extrap_method=simscape.enum.extrapolation.nearest
  ExtWall (A3R2W1) : ExternalWall_lib/Wall External  extWallModel=wallExternalModelOption.wallSolarWin  wallLength=4.2672 % Parameterized on : 13-Jun-2026 10:47:12 m  wallHeight=3.048 % Parameterized on : 13-Jun-2026 10:47:12 m  wallThickness=0.07 % Parameterized on : 13-Jun-2026 10:47:12 m  wallMaterialDen=2000 % Parameterized on : 13-Jun-2026 10:47:17 kg/m^3  wallMaterialCp=1100 % Parameterized on : 13-Jun-2026 10:47:17 J/(K*kg)  wallAbsorptivity=0.6 % Parameterized on : 13-Jun-2026 10:47:17  wallThermalK=1.4 % Parameterized on : 13-Jun-2026 10:47:17 W/(K*m)  winLength=3.3054 % Parameterized on : 13-Jun-2026 10:47:12 m  winHeight=2.361 % Parameterized on : 13-Jun-2026 10:47:12 m  winThickness=0.005 % Parameterized on : 13-Jun-2026 10:47:17 m  winMaterialDen=4000 % Parameterized on : 13-Jun-2026 10:47:17 kg/m^3  winMaterialCp=840 % Parameterized on : 13-Jun-2026 10:47:17 J/(K*kg)  winAbsorptivity=0.4 % Parameterized on : 13-Jun-2026 10:47:17  winThermalK=1 % Parameterized on : 13-Jun-2026 10:47:17 W/(K*m)  winTransmissivity=0.2 % Parameterized on : 13-Jun-2026 10:47:17  ventLength=0.1 m  ventHeight=0.1 m  extToWallHTC=20 % Parameterized on : 13-Jun-2026 10:47:17 W/(K*m^2)  intToRoomHTC=30 % Parameterized on : 13-Jun-2026 10:47:17 W/(K*m^2)  iniT=300 % Parameterized on : 13-Jun-2026 10:47:17 K  latitude=5  longitude=5  localTime=5  dayLightS=0  surfAngle=90 % Parameterized on : 13-Jun-2026 10:47:12 deg  surfUnitV="[0  1] % Parameterized on : 13-Jun-2026 10:47:12"  startYear=2025  startMonth=1  startDay=1  startHr=1  numHrsData=24  interp_method=simscape.enum.interpolation.linear  extrap_method=simscape.enum.extrapolation.nearest
  ExtWall (A3R2W2) : ExternalWall_lib/Wall External  extWallModel=wallExternalModelOption.wallSolar  wallLength=4.572 % Parameterized on : 13-Jun-2026 10:47:12 m  wallHeight=3.048 % Parameterized on : 13-Jun-2026 10:47:12 m  wallThickness=0.07 % Parameterized on : 13-Jun-2026 10:47:12 m  wallMaterialDen=2000 % Parameterized on : 13-Jun-2026 10:47:17 kg/m^3  wallMaterialCp=1100 % Parameterized on : 13-Jun-2026 10:47:17 J/(K*kg)  wallAbsorptivity=0.6 % Parameterized on : 13-Jun-2026 10:47:17  wallThermalK=1.4 % Parameterized on : 13-Jun-2026 10:47:17 W/(K*m)  winLength=1 m  winHeight=0.5 m  winThickness=0.007 m  winMaterialDen=2500 kg/m^3  winMaterialCp=787 J/(K*kg)  winAbsorptivity=0.35  winThermalK=1 W/(K*m)  winTransmissivity=0.45  ventLength=0.1 m  ventHeight=0.1 m  extToWallHTC=20 % Parameterized on : 13-Jun-2026 10:47:17 W/(K*m^2)  intToRoomHTC=30 % Parameterized on : 13-Jun-2026 10:47:17 W/(K*m^2)  iniT=300 % Parameterized on : 13-Jun-2026 10:47:17 K  latitude=5  longitude=5  localTime=5  dayLightS=0  surfAngle=90 % Parameterized on : 13-Jun-2026 10:47:12 deg  surfUnitV="[1  0] % Parameterized on : 13-Jun-2026 10:47:12"  startYear=2025  startMonth=1  startDay=1  startHr=1  numHrsData=24  interp_method=simscape.enum.interpolation.linear  extrap_method=simscape.enum.extrapolation.nearest
  ExtWall (A3R2W3) : ExternalWall_lib/Wall External  extWallModel=wallExternalModelOption.wallSolarWin  wallLength=4.2672 % Parameterized on : 13-Jun-2026 10:47:12 m  wallHeight=3.048 % Parameterized on : 13-Jun-2026 10:47:12 m  wallThickness=0.07 % Parameterized on : 13-Jun-2026 10:47:12 m  wallMaterialDen=2000 % Parameterized on : 13-Jun-2026 10:47:17 kg/m^3  wallMaterialCp=1100 % Parameterized on : 13-Jun-2026 10:47:17 J/(K*kg)  wallAbsorptivity=0.6 % Parameterized on : 13-Jun-2026 10:47:17  wallThermalK=1.4 % Parameterized on : 13-Jun-2026 10:47:17 W/(K*m)  winLength=3.8167 % Parameterized on : 13-Jun-2026 10:47:12 m  winHeight=2.7262 % Parameterized on : 13-Jun-2026 10:47:12 m  winThickness=0.005 % Parameterized on : 13-Jun-2026 10:47:17 m  winMaterialDen=4000 % Parameterized on : 13-Jun-2026 10:47:17 kg/m^3  winMaterialCp=840 % Parameterized on : 13-Jun-2026 10:47:17 J/(K*kg)  winAbsorptivity=0.4 % Parameterized on : 13-Jun-2026 10:47:17  winThermalK=1 % Parameterized on : 13-Jun-2026 10:47:17 W/(K*m)  winTransmissivity=0.2 % Parameterized on : 13-Jun-2026 10:47:17  ventLength=0.1 m  ventHeight=0.1 m  extToWallHTC=20 % Parameterized on : 13-Jun-2026 10:47:17 W/(K*m^2)  intToRoomHTC=30 % Parameterized on : 13-Jun-2026 10:47:17 W/(K*m^2)  iniT=300 % Parameterized on : 13-Jun-2026 10:47:17 K  latitude=5  longitude=5  localTime=5  dayLightS=0  surfAngle=90 % Parameterized on : 13-Jun-2026 10:47:12 deg  surfUnitV=[0 -1] % Parameterized on : 13-Jun-2026 10:47:12  startYear=2025  startMonth=1  startDay=1  startHr=1  numHrsData=24  interp_method=simscape.enum.interpolation.linear  extrap_method=simscape.enum.extrapolation.nearest
  ExtWall (A3R3W1) : ExternalWall_lib/Wall External  extWallModel=wallExternalModelOption.wallSolarWin  wallLength=2.7432 % Parameterized on : 13-Jun-2026 10:47:12 m  wallHeight=3.048 % Parameterized on : 13-Jun-2026 10:47:12 m  wallThickness=0.07 % Parameterized on : 13-Jun-2026 10:47:12 m  wallMaterialDen=2000 % Parameterized on : 13-Jun-2026 10:47:17 kg/m^3  wallMaterialCp=1100 % Parameterized on : 13-Jun-2026 10:47:17 J/(K*kg)  wallAbsorptivity=0.6 % Parameterized on : 13-Jun-2026 10:47:17  wallThermalK=1.4 % Parameterized on : 13-Jun-2026 10:47:17 W/(K*m)  winLength=1.9397 % Parameterized on : 13-Jun-2026 10:47:12 m  winHeight=2.1553 % Parameterized on : 13-Jun-2026 10:47:12 m  winThickness=0.005 % Parameterized on : 13-Jun-2026 10:47:17 m  winMaterialDen=4000 % Parameterized on : 13-Jun-2026 10:47:17 kg/m^3  winMaterialCp=840 % Parameterized on : 13-Jun-2026 10:47:17 J/(K*kg)  winAbsorptivity=0.4 % Parameterized on : 13-Jun-2026 10:47:17  winThermalK=1 % Parameterized on : 13-Jun-2026 10:47:17 W/(K*m)  winTransmissivity=0.2 % Parameterized on : 13-Jun-2026 10:47:17  ventLength=0.1 m  ventHeight=0.1 m  extToWallHTC=20 % Parameterized on : 13-Jun-2026 10:47:17 W/(K*m^2)  intToRoomHTC=30 % Parameterized on : 13-Jun-2026 10:47:17 W/(K*m^2)  iniT=300 % Parameterized on : 13-Jun-2026 10:47:17 K  latitude=5  longitude=5  localTime=5  dayLightS=0  surfAngle=90 % Parameterized on : 13-Jun-2026 10:47:12 deg  surfUnitV="[-1  0] % Parameterized on : 13-Jun-2026 10:47:12"  startYear=2025  startMonth=1  startDay=1  startHr=1  numHrsData=24  interp_method=simscape.enum.interpolation.linear  extrap_method=simscape.enum.extrapolation.nearest
  ExtWall (A3R3W2) : ExternalWall_lib/Wall External  extWallModel=wallExternalModelOption.wallSolarWin  wallLength=3.9624 % Parameterized on : 13-Jun-2026 10:47:12 m  wallHeight=3.048 % Parameterized on : 13-Jun-2026 10:47:12 m  wallThickness=0.07 % Parameterized on : 13-Jun-2026 10:47:12 m  wallMaterialDen=2000 % Parameterized on : 13-Jun-2026 10:47:17 kg/m^3  wallMaterialCp=1100 % Parameterized on : 13-Jun-2026 10:47:17 J/(K*kg)  wallAbsorptivity=0.6 % Parameterized on : 13-Jun-2026 10:47:18  wallThermalK=1.4 % Parameterized on : 13-Jun-2026 10:47:18 W/(K*m)  winLength=2.8018 % Parameterized on : 13-Jun-2026 10:47:12 m  winHeight=2.1553 % Parameterized on : 13-Jun-2026 10:47:12 m  winThickness=0.005 % Parameterized on : 13-Jun-2026 10:47:18 m  winMaterialDen=4000 % Parameterized on : 13-Jun-2026 10:47:18 kg/m^3  winMaterialCp=840 % Parameterized on : 13-Jun-2026 10:47:18 J/(K*kg)  winAbsorptivity=0.4 % Parameterized on : 13-Jun-2026 10:47:18  winThermalK=1 % Parameterized on : 13-Jun-2026 10:47:18 W/(K*m)  winTransmissivity=0.2 % Parameterized on : 13-Jun-2026 10:47:18  ventLength=0.1 m  ventHeight=0.1 m  extToWallHTC=20 % Parameterized on : 13-Jun-2026 10:47:18 W/(K*m^2)  intToRoomHTC=30 % Parameterized on : 13-Jun-2026 10:47:18 W/(K*m^2)  iniT=300 % Parameterized on : 13-Jun-2026 10:47:18 K  latitude=5  longitude=5  localTime=5  dayLightS=0  surfAngle=90 % Parameterized on : 13-Jun-2026 10:47:12 deg  surfUnitV="[0  1] % Parameterized on : 13-Jun-2026 10:47:12"  startYear=2025  startMonth=1  startDay=1  startHr=1  numHrsData=24  interp_method=simscape.enum.interpolation.linear  extrap_method=simscape.enum.extrapolation.nearest
  ExtWall (A3R3W3) : ExternalWall_lib/Wall External  extWallModel=wallExternalModelOption.wallSolar  wallLength=2.7432 % Parameterized on : 13-Jun-2026 10:47:12 m  wallHeight=3.048 % Parameterized on : 13-Jun-2026 10:47:12 m  wallThickness=0.07 % Parameterized on : 13-Jun-2026 10:47:12 m  wallMaterialDen=2000 % Parameterized on : 13-Jun-2026 10:47:18 kg/m^3  wallMaterialCp=1100 % Parameterized on : 13-Jun-2026 10:47:18 J/(K*kg)  wallAbsorptivity=0.6 % Parameterized on : 13-Jun-2026 10:47:18  wallThermalK=1.4 % Parameterized on : 13-Jun-2026 10:47:18 W/(K*m)  winLength=1 m  winHeight=0.5 m  winThickness=0.007 m  winMaterialDen=2500 kg/m^3  winMaterialCp=787 J/(K*kg)  winAbsorptivity=0.35  winThermalK=1 W/(K*m)  winTransmissivity=0.45  ventLength=0.1 m  ventHeight=0.1 m  extToWallHTC=20 % Parameterized on : 13-Jun-2026 10:47:18 W/(K*m^2)  intToRoomHTC=30 % Parameterized on : 13-Jun-2026 10:47:18 W/(K*m^2)  iniT=300 % Parameterized on : 13-Jun-2026 10:47:18 K  latitude=5  longitude=5  localTime=5  dayLightS=0  surfAngle=90 % Parameterized on : 13-Jun-2026 10:47:12 deg  surfUnitV="[1  0] % Parameterized on : 13-Jun-2026 10:47:12"  startYear=2025  startMonth=1  startDay=1  startHr=1  numHrsData=24  interp_method=simscape.enum.interpolation.linear  extrap_method=simscape.enum.extrapolation.nearest
  ExtWall (A3R4W3) : ExternalWall_lib/Wall External  extWallModel=wallExternalModelOption.wallSolar  wallLength=2.4384 % Parameterized on : 13-Jun-2026 10:47:12 m  wallHeight=3.048 % Parameterized on : 13-Jun-2026 10:47:12 m  wallThickness=0.07 % Parameterized on : 13-Jun-2026 10:47:12 m  wallMaterialDen=2000 % Parameterized on : 13-Jun-2026 10:47:18 kg/m^3  wallMaterialCp=1100 % Parameterized on : 13-Jun-2026 10:47:18 J/(K*kg)  wallAbsorptivity=0.6 % Parameterized on : 13-Jun-2026 10:47:18  wallThermalK=1.4 % Parameterized on : 13-Jun-2026 10:47:18 W/(K*m)  winLength=1 m  winHeight=0.5 m  winThickness=0.007 m  winMaterialDen=2500 kg/m^3  winMaterialCp=787 J/(K*kg)  winAbsorptivity=0.35  winThermalK=1 W/(K*m)  winTransmissivity=0.45  ventLength=0.1 m  ventHeight=0.1 m  extToWallHTC=20 % Parameterized on : 13-Jun-2026 10:47:18 W/(K*m^2)  intToRoomHTC=30 % Parameterized on : 13-Jun-2026 10:47:18 W/(K*m^2)  iniT=300 % Parameterized on : 13-Jun-2026 10:47:18 K  latitude=5  longitude=5  localTime=5  dayLightS=0  surfAngle=90 % Parameterized on : 13-Jun-2026 10:47:12 deg  surfUnitV="[1  0] % Parameterized on : 13-Jun-2026 10:47:12"  startYear=2025  startMonth=1  startDay=1  startHr=1  numHrsData=24  interp_method=simscape.enum.interpolation.linear  extrap_method=simscape.enum.extrapolation.nearest
  ExtWall (A3R5W2) : ExternalWall_lib/Wall External  extWallModel=wallExternalModelOption.wallSolar  wallLength=2.1336 % Parameterized on : 13-Jun-2026 10:47:12 m  wallHeight=3.048 % Parameterized on : 13-Jun-2026 10:47:12 m  wallThickness=0.07 % Parameterized on : 13-Jun-2026 10:47:12 m  wallMaterialDen=2000 % Parameterized on : 13-Jun-2026 10:47:18 kg/m^3  wallMaterialCp=1100 % Parameterized on : 13-Jun-2026 10:47:18 J/(K*kg)  wallAbsorptivity=0.6 % Parameterized on : 13-Jun-2026 10:47:18  wallThermalK=1.4 % Parameterized on : 13-Jun-2026 10:47:18 W/(K*m)  winLength=1 m  winHeight=0.5 m  winThickness=0.007 m  winMaterialDen=2500 kg/m^3  winMaterialCp=787 J/(K*kg)  winAbsorptivity=0.35  winThermalK=1 W/(K*m)  winTransmissivity=0.45  ventLength=0.1 m  ventHeight=0.1 m  extToWallHTC=20 % Parameterized on : 13-Jun-2026 10:47:18 W/(K*m^2)  intToRoomHTC=30 % Parameterized on : 13-Jun-2026 10:47:18 W/(K*m^2)  iniT=300 % Parameterized on : 13-Jun-2026 10:47:18 K  latitude=5  longitude=5  localTime=5  dayLightS=0  surfAngle=90 % Parameterized on : 13-Jun-2026 10:47:12 deg  surfUnitV="[-6.0708e-17           1] % Parameterized on : 13-Jun-2026 10:47:12"  startYear=2025  startMonth=1  startDay=1  startHr=1  numHrsData=24  interp_method=simscape.enum.interpolation.linear  extrap_method=simscape.enum.extrapolation.nearest
  ExtWall (A4R2W1) : ExternalWall_lib/Wall External  extWallModel=wallExternalModelOption.wallSolarWin  wallLength=4.2672 % Parameterized on : 13-Jun-2026 10:47:12 m  wallHeight=3.048 % Parameterized on : 13-Jun-2026 10:47:12 m  wallThickness=0.07 % Parameterized on : 13-Jun-2026 10:47:12 m  wallMaterialDen=2000 % Parameterized on : 13-Jun-2026 10:47:18 kg/m^3  wallMaterialCp=1100 % Parameterized on : 13-Jun-2026 10:47:18 J/(K*kg)  wallAbsorptivity=0.6 % Parameterized on : 13-Jun-2026 10:47:18  wallThermalK=1.4 % Parameterized on : 13-Jun-2026 10:47:18 W/(K*m)  winLength=3.0174 % Parameterized on : 13-Jun-2026 10:47:12 m  winHeight=2.1553 % Parameterized on : 13-Jun-2026 10:47:12 m  winThickness=0.005 % Parameterized on : 13-Jun-2026 10:47:18 m  winMaterialDen=4000 % Parameterized on : 13-Jun-2026 10:47:18 kg/m^3  winMaterialCp=840 % Parameterized on : 13-Jun-2026 10:47:18 J/(K*kg)  winAbsorptivity=0.4 % Parameterized on : 13-Jun-2026 10:47:18  winThermalK=1 % Parameterized on : 13-Jun-2026 10:47:18 W/(K*m)  winTransmissivity=0.2 % Parameterized on : 13-Jun-2026 10:47:18  ventLength=0.1 m  ventHeight=0.1 m  extToWallHTC=20 % Parameterized on : 13-Jun-2026 10:47:18 W/(K*m^2)  intToRoomHTC=30 % Parameterized on : 13-Jun-2026 10:47:18 W/(K*m^2)  iniT=300 % Parameterized on : 13-Jun-2026 10:47:18 K  latitude=5  longitude=5  localTime=5  dayLightS=0  surfAngle=90 % Parameterized on : 13-Jun-2026 10:47:12 deg  surfUnitV="[0  1] % Parameterized on : 13-Jun-2026 10:47:12"  startYear=2025  startMonth=1  startDay=1  startHr=1  numHrsData=24  interp_method=simscape.enum.interpolation.linear  extrap_method=simscape.enum.extrapolation.nearest
  ExtWall (A4R2W3) : ExternalWall_lib/Wall External  extWallModel=wallExternalModelOption.wallSolarWin  wallLength=4.2672 % Parameterized on : 13-Jun-2026 10:47:12 m  wallHeight=3.048 % Parameterized on : 13-Jun-2026 10:47:12 m  wallThickness=0.07 % Parameterized on : 13-Jun-2026 10:47:12 m  wallMaterialDen=2000 % Parameterized on : 13-Jun-2026 10:47:18 kg/m^3  wallMaterialCp=1100 % Parameterized on : 13-Jun-2026 10:47:18 J/(K*kg)  wallAbsorptivity=0.6 % Parameterized on : 13-Jun-2026 10:47:18  wallThermalK=1.4 % Parameterized on : 13-Jun-2026 10:47:18 W/(K*m)  winLength=3.3054 % Parameterized on : 13-Jun-2026 10:47:12 m  winHeight=2.361 % Parameterized on : 13-Jun-2026 10:47:12 m  winThickness=0.005 % Parameterized on : 13-Jun-2026 10:47:18 m  winMaterialDen=4000 % Parameterized on : 13-Jun-2026 10:47:18 kg/m^3  winMaterialCp=840 % Parameterized on : 13-Jun-2026 10:47:18 J/(K*kg)  winAbsorptivity=0.4 % Parameterized on : 13-Jun-2026 10:47:18  winThermalK=1 % Parameterized on : 13-Jun-2026 10:47:18 W/(K*m)  winTransmissivity=0.2 % Parameterized on : 13-Jun-2026 10:47:18  ventLength=0.1 m  ventHeight=0.1 m  extToWallHTC=20 % Parameterized on : 13-Jun-2026 10:47:18 W/(K*m^2)  intToRoomHTC=30 % Parameterized on : 13-Jun-2026 10:47:18 W/(K*m^2)  iniT=300 % Parameterized on : 13-Jun-2026 10:47:18 K  latitude=5  longitude=5  localTime=5  dayLightS=0  surfAngle=90 % Parameterized on : 13-Jun-2026 10:47:12 deg  surfUnitV=[0 -1] % Parameterized on : 13-Jun-2026 10:47:12  startYear=2025  startMonth=1  startDay=1  startHr=1  numHrsData=24  interp_method=simscape.enum.interpolation.linear  extrap_method=simscape.enum.extrapolation.nearest
  ExtWall (A4R2W4) : ExternalWall_lib/Wall External  extWallModel=wallExternalModelOption.wallSolar  wallLength=4.572 % Parameterized on : 13-Jun-2026 10:47:12 m  wallHeight=3.048 % Parameterized on : 13-Jun-2026 10:47:12 m  wallThickness=0.07 % Parameterized on : 13-Jun-2026 10:47:12 m  wallMaterialDen=2000 % Parameterized on : 13-Jun-2026 10:47:18 kg/m^3  wallMaterialCp=1100 % Parameterized on : 13-Jun-2026 10:47:18 J/(K*kg)  wallAbsorptivity=0.6 % Parameterized on : 13-Jun-2026 10:47:18  wallThermalK=1.4 % Parameterized on : 13-Jun-2026 10:47:18 W/(K*m)  winLength=1 m  winHeight=0.5 m  winThickness=0.007 m  winMaterialDen=2500 kg/m^3  winMaterialCp=787 J/(K*kg)  winAbsorptivity=0.35  winThermalK=1 W/(K*m)  winTransmissivity=0.45  ventLength=0.1 m  ventHeight=0.1 m  extToWallHTC=20 % Parameterized on : 13-Jun-2026 10:47:18 W/(K*m^2)  intToRoomHTC=30 % Parameterized on : 13-Jun-2026 10:47:18 W/(K*m^2)  iniT=300 % Parameterized on : 13-Jun-2026 10:47:18 K  latitude=5  longitude=5  localTime=5  dayLightS=0  surfAngle=90 % Parameterized on : 13-Jun-2026 10:47:12 deg  surfUnitV="[-1  0] % Parameterized on : 13-Jun-2026 10:47:12"  startYear=2025  startMonth=1  startDay=1  startHr=1  numHrsData=24  interp_method=simscape.enum.interpolation.linear  extrap_method=simscape.enum.extrapolation.nearest
  ExtWall (A4R3W1) : ExternalWall_lib/Wall External  extWallModel=wallExternalModelOption.wallSolarWin  wallLength=2.7432 % Parameterized on : 13-Jun-2026 10:47:12 m  wallHeight=3.048 % Parameterized on : 13-Jun-2026 10:47:12 m  wallThickness=0.07 % Parameterized on : 13-Jun-2026 10:47:12 m  wallMaterialDen=2000 % Parameterized on : 13-Jun-2026 10:47:18 kg/m^3  wallMaterialCp=1100 % Parameterized on : 13-Jun-2026 10:47:18 J/(K*kg)  wallAbsorptivity=0.6 % Parameterized on : 13-Jun-2026 10:47:18  wallThermalK=1.4 % Parameterized on : 13-Jun-2026 10:47:18 W/(K*m)  winLength=2.4536 % Parameterized on : 13-Jun-2026 10:47:12 m  winHeight=2.7262 % Parameterized on : 13-Jun-2026 10:47:12 m  winThickness=0.005 % Parameterized on : 13-Jun-2026 10:47:18 m  winMaterialDen=4000 % Parameterized on : 13-Jun-2026 10:47:18 kg/m^3  winMaterialCp=840 % Parameterized on : 13-Jun-2026 10:47:18 J/(K*kg)  winAbsorptivity=0.4 % Parameterized on : 13-Jun-2026 10:47:18  winThermalK=1 % Parameterized on : 13-Jun-2026 10:47:18 W/(K*m)  winTransmissivity=0.2 % Parameterized on : 13-Jun-2026 10:47:18  ventLength=0.1 m  ventHeight=0.1 m  extToWallHTC=20 % Parameterized on : 13-Jun-2026 10:47:18 W/(K*m^2)  intToRoomHTC=30 % Parameterized on : 13-Jun-2026 10:47:18 W/(K*m^2)  iniT=300 % Parameterized on : 13-Jun-2026 10:47:18 K  latitude=5  longitude=5  localTime=5  dayLightS=0  surfAngle=90 % Parameterized on : 13-Jun-2026 10:47:12 deg  surfUnitV="[1  0] % Parameterized on : 13-Jun-2026 10:47:12"  startYear=2025  startMonth=1  startDay=1  startHr=1  numHrsData=24  interp_method=simscape.enum.interpolation.linear  extrap_method=simscape.enum.extrapolation.nearest
  ExtWall (A4R3W3) : ExternalWall_lib/Wall External  extWallModel=wallExternalModelOption.wallSolarWin  wallLength=2.7432 % Parameterized on : 13-Jun-2026 10:47:12 m  wallHeight=3.048 % Parameterized on : 13-Jun-2026 10:47:12 m  wallThickness=0.07 % Parameterized on : 13-Jun-2026 10:47:12 m  wallMaterialDen=2000 % Parameterized on : 13-Jun-2026 10:47:18 kg/m^3  wallMaterialCp=1100 % Parameterized on : 13-Jun-2026 10:47:18 J/(K*kg)  wallAbsorptivity=0.6 % Parameterized on : 13-Jun-2026 10:47:18  wallThermalK=1.4 % Parameterized on : 13-Jun-2026 10:47:18 W/(K*m)  winLength=1.9397 % Parameterized on : 13-Jun-2026 10:47:12 m  winHeight=2.1553 % Parameterized on : 13-Jun-2026 10:47:12 m  winThickness=0.005 % Parameterized on : 13-Jun-2026 10:47:18 m  winMaterialDen=4000 % Parameterized on : 13-Jun-2026 10:47:18 kg/m^3  winMaterialCp=840 % Parameterized on : 13-Jun-2026 10:47:18 J/(K*kg)  winAbsorptivity=0.4 % Parameterized on : 13-Jun-2026 10:47:18  winThermalK=1 % Parameterized on : 13-Jun-2026 10:47:18 W/(K*m)  winTransmissivity=0.2 % Parameterized on : 13-Jun-2026 10:47:18  ventLength=0.1 m  ventHeight=0.1 m  extToWallHTC=20 % Parameterized on : 13-Jun-2026 10:47:18 W/(K*m^2)  intToRoomHTC=30 % Parameterized on : 13-Jun-2026 10:47:18 W/(K*m^2)  iniT=300 % Parameterized on : 13-Jun-2026 10:47:18 K  latitude=5  longitude=5  localTime=5  dayLightS=0  surfAngle=90 % Parameterized on : 13-Jun-2026 10:47:12 deg  surfUnitV="[-1  0] % Parameterized on : 13-Jun-2026 10:47:12"  startYear=2025  startMonth=1  startDay=1  startHr=1  numHrsData=24  interp_method=simscape.enum.interpolation.linear  extrap_method=simscape.enum.extrapolation.nearest
  ExtWall (A4R3W4) : ExternalWall_lib/Wall External  extWallModel=wallExternalModelOption.wallSolar  wallLength=3.9624 % Parameterized on : 13-Jun-2026 10:47:12 m  wallHeight=3.048 % Parameterized on : 13-Jun-2026 10:47:12 m  wallThickness=0.07 % Parameterized on : 13-Jun-2026 10:47:12 m  wallMaterialDen=2000 % Parameterized on : 13-Jun-2026 10:47:18 kg/m^3  wallMaterialCp=1100 % Parameterized on : 13-Jun-2026 10:47:18 J/(K*kg)  wallAbsorptivity=0.6 % Parameterized on : 13-Jun-2026 10:47:18  wallThermalK=1.4 % Parameterized on : 13-Jun-2026 10:47:18 W/(K*m)  winLength=1 m  winHeight=0.5 m  winThickness=0.007 m  winMaterialDen=2500 kg/m^3  winMaterialCp=787 J/(K*kg)  winAbsorptivity=0.35  winThermalK=1 W/(K*m)  winTransmissivity=0.45  ventLength=0.1 m  ventHeight=0.1 m  extToWallHTC=20 % Parameterized on : 13-Jun-2026 10:47:18 W/(K*m^2)  intToRoomHTC=30 % Parameterized on : 13-Jun-2026 10:47:18 W/(K*m^2)  iniT=300 % Parameterized on : 13-Jun-2026 10:47:18 K  latitude=5  longitude=5  localTime=5  dayLightS=0  surfAngle=90 % Parameterized on : 13-Jun-2026 10:47:12 deg  surfUnitV="[0  1] % Parameterized on : 13-Jun-2026 10:47:12"  startYear=2025  startMonth=1  startDay=1  startHr=1  numHrsData=24  interp_method=simscape.enum.interpolation.linear  extrap_method=simscape.enum.extrapolation.nearest
  ExtWall (A4R4W3) : ExternalWall_lib/Wall External  extWallModel=wallExternalModelOption.wallSolar  wallLength=2.4384 % Parameterized on : 13-Jun-2026 10:47:12 m  wallHeight=3.048 % Parameterized on : 13-Jun-2026 10:47:12 m  wallThickness=0.07 % Parameterized on : 13-Jun-2026 10:47:12 m  wallMaterialDen=2000 % Parameterized on : 13-Jun-2026 10:47:18 kg/m^3  wallMaterialCp=1100 % Parameterized on : 13-Jun-2026 10:47:18 J/(K*kg)  wallAbsorptivity=0.6 % Parameterized on : 13-Jun-2026 10:47:18  wallThermalK=1.4 % Parameterized on : 13-Jun-2026 10:47:18 W/(K*m)  winLength=1 m  winHeight=0.5 m  winThickness=0.007 m  winMaterialDen=2500 kg/m^3  winMaterialCp=787 J/(K*kg)  winAbsorptivity=0.35  winThermalK=1 W/(K*m)  winTransmissivity=0.45  ventLength=0.1 m  ventHeight=0.1 m  extToWallHTC=20 % Parameterized on : 13-Jun-2026 10:47:18 W/(K*m^2)  intToRoomHTC=30 % Parameterized on : 13-Jun-2026 10:47:18 W/(K*m^2)  iniT=300 % Parameterized on : 13-Jun-2026 10:47:18 K  latitude=5  longitude=5  localTime=5  dayLightS=0  surfAngle=90 % Parameterized on : 13-Jun-2026 10:47:12 deg  surfUnitV="[-1  4.8566e-16] % Parameterized on : 13-Jun-2026 10:47:12"  startYear=2025  startMonth=1  startDay=1  startHr=1  numHrsData=24  interp_method=simscape.enum.interpolation.linear  extrap_method=simscape.enum.extrapolation.nearest
  ExtWall (A4R5W4) : ExternalWall_lib/Wall External  extWallModel=wallExternalModelOption.wallSolar  wallLength=2.1336 % Parameterized on : 13-Jun-2026 10:47:12 m  wallHeight=3.048 % Parameterized on : 13-Jun-2026 10:47:12 m  wallThickness=0.07 % Parameterized on : 13-Jun-2026 10:47:12 m  wallMaterialDen=2000 % Parameterized on : 13-Jun-2026 10:47:18 kg/m^3  wallMaterialCp=1100 % Parameterized on : 13-Jun-2026 10:47:18 J/(K*kg)  wallAbsorptivity=0.6 % Parameterized on : 13-Jun-2026 10:47:18  wallThermalK=1.4 % Parameterized on : 13-Jun-2026 10:47:18 W/(K*m)  winLength=1 m  winHeight=0.5 m  winThickness=0.007 m  winMaterialDen=2500 kg/m^3  winMaterialCp=787 J/(K*kg)  winAbsorptivity=0.35  winThermalK=1 W/(K*m)  winTransmissivity=0.45  ventLength=0.1 m  ventHeight=0.1 m  extToWallHTC=20 % Parameterized on : 13-Jun-2026 10:47:18 W/(K*m^2)  intToRoomHTC=30 % Parameterized on : 13-Jun-2026 10:47:18 W/(K*m^2)  iniT=300 % Parameterized on : 13-Jun-2026 10:47:18 K  latitude=5  longitude=5  localTime=5  dayLightS=0  surfAngle=90 % Parameterized on : 13-Jun-2026 10:47:12 deg  surfUnitV="[0  1] % Parameterized on : 13-Jun-2026 10:47:12"  startYear=2025  startMonth=1  startDay=1  startHr=1  numHrsData=24  interp_method=simscape.enum.interpolation.linear  extrap_method=simscape.enum.extrapolation.nearest
  Room_A1R1_LivingRoom_A : RoomWithAirVolume/Room with Air Volume  roomWid=4.572 % Parameterized on : 13-Jun-2026 10:47:11  roomHgt=3.048 % Parameterized on : 13-Jun-2026 10:47:11  roomLen=2.4384 % Parameterized on : 13-Jun-2026 10:47:11  htc=30 % Parameterized on : 13-Jun-2026 10:47:16  iniT=300 % Parameterized on : 13-Jun-2026 10:47:16  indxS=1
  Room_A1R2_Bedroom_A : RoomWithAirVolume/Room with Air Volume  roomWid=4.572 % Parameterized on : 13-Jun-2026 10:47:11  roomHgt=3.048 % Parameterized on : 13-Jun-2026 10:47:11  roomLen=4.2672 % Parameterized on : 13-Jun-2026 10:47:11  htc=30 % Parameterized on : 13-Jun-2026 10:47:16  iniT=300 % Parameterized on : 13-Jun-2026 10:47:16  indxS=2
  Room_A1R3_Kitchen_A : RoomWithAirVolume/Room with Air Volume  roomWid=3.9624 % Parameterized on : 13-Jun-2026 10:47:11  roomHgt=3.048 % Parameterized on : 13-Jun-2026 10:47:11  roomLen=2.7432 % Parameterized on : 13-Jun-2026 10:47:11  htc=30 % Parameterized on : 13-Jun-2026 10:47:16  iniT=300 % Parameterized on : 13-Jun-2026 10:47:16  indxS=3
  Room_A1R4_Bathroom_A : RoomWithAirVolume/Room with Air Volume  roomWid=3.6576 % Parameterized on : 13-Jun-2026 10:47:11  roomHgt=3.048 % Parameterized on : 13-Jun-2026 10:47:11  roomLen=2.4384 % Parameterized on : 13-Jun-2026 10:47:11  htc=30 % Parameterized on : 13-Jun-2026 10:47:16  iniT=300 % Parameterized on : 13-Jun-2026 10:47:16  indxS=4
  Room_A1R5_FireExit_A : RoomWithAirVolume/Room with Air Volume  roomWid=2.1336 % Parameterized on : 13-Jun-2026 10:47:11  roomHgt=3.048 % Parameterized on : 13-Jun-2026 10:47:11  roomLen=1.8288 % Parameterized on : 13-Jun-2026 10:47:11  htc=30 % Parameterized on : 13-Jun-2026 10:47:16  iniT=300 % Parameterized on : 13-Jun-2026 10:47:16  indxS=5
  Room_A1R6_Lobby1_A : RoomWithAirVolume/Room with Air Volume  roomWid=2.4384 % Parameterized on : 13-Jun-2026 10:47:11  roomHgt=3.048 % Parameterized on : 13-Jun-2026 10:47:11  roomLen=2.4384 % Parameterized on : 13-Jun-2026 10:47:11  htc=30 % Parameterized on : 13-Jun-2026 10:47:16  iniT=300 % Parameterized on : 13-Jun-2026 10:47:16  indxS=6
  Room_A1R7_Lobby2_A : RoomWithAirVolume/Room with Air Volume  roomWid=1.524 % Parameterized on : 13-Jun-2026 10:47:11  roomHgt=3.048 % Parameterized on : 13-Jun-2026 10:47:11  roomLen=2.4384 % Parameterized on : 13-Jun-2026 10:47:11  htc=30 % Parameterized on : 13-Jun-2026 10:47:16  iniT=300 % Parameterized on : 13-Jun-2026 10:47:16  indxS=7
  Room_A2R1_LivingRoom_B : RoomWithAirVolume/Room with Air Volume  roomWid=4.572 % Parameterized on : 13-Jun-2026 10:47:11  roomHgt=3.048 % Parameterized on : 13-Jun-2026 10:47:11  roomLen=2.4384 % Parameterized on : 13-Jun-2026 10:47:11  htc=30 % Parameterized on : 13-Jun-2026 10:47:16  iniT=300 % Parameterized on : 13-Jun-2026 10:47:16  indxS=8
  Room_A2R2_Bedroom_B : RoomWithAirVolume/Room with Air Volume  roomWid=4.572 % Parameterized on : 13-Jun-2026 10:47:11  roomHgt=3.048 % Parameterized on : 13-Jun-2026 10:47:11  roomLen=4.2672 % Parameterized on : 13-Jun-2026 10:47:11  htc=30 % Parameterized on : 13-Jun-2026 10:47:16  iniT=300 % Parameterized on : 13-Jun-2026 10:47:16  indxS=9
  Room_A2R3_Kitchen_B : RoomWithAirVolume/Room with Air Volume  roomWid=3.9624 % Parameterized on : 13-Jun-2026 10:47:11  roomHgt=3.048 % Parameterized on : 13-Jun-2026 10:47:11  roomLen=2.7432 % Parameterized on : 13-Jun-2026 10:47:11  htc=30 % Parameterized on : 13-Jun-2026 10:47:16  iniT=300 % Parameterized on : 13-Jun-2026 10:47:16  indxS=10
  Room_A2R4_Bathroom_B : RoomWithAirVolume/Room with Air Volume  roomWid=3.6576 % Parameterized on : 13-Jun-2026 10:47:11  roomHgt=3.048 % Parameterized on : 13-Jun-2026 10:47:11  roomLen=2.4384 % Parameterized on : 13-Jun-2026 10:47:11  htc=30 % Parameterized on : 13-Jun-2026 10:47:16  iniT=300 % Parameterized on : 13-Jun-2026 10:47:16  indxS=11
  Room_A2R5_FireExit_B : RoomWithAirVolume/Room with Air Volume  roomWid=2.1336 % Parameterized on : 13-Jun-2026 10:47:11  roomHgt=3.048 % Parameterized on : 13-Jun-2026 10:47:11  roomLen=1.8288 % Parameterized on : 13-Jun-2026 10:47:11  htc=30 % Parameterized on : 13-Jun-2026 10:47:16  iniT=300 % Parameterized on : 13-Jun-2026 10:47:16  indxS=12
  Room_A2R6_Lobby1_B : RoomWithAirVolume/Room with Air Volume  roomWid=2.4384 % Parameterized on : 13-Jun-2026 10:47:11  roomHgt=3.048 % Parameterized on : 13-Jun-2026 10:47:11  roomLen=2.4384 % Parameterized on : 13-Jun-2026 10:47:11  htc=30 % Parameterized on : 13-Jun-2026 10:47:16  iniT=300 % Parameterized on : 13-Jun-2026 10:47:16  indxS=13
  Room_A2R7_Lobby2_B : RoomWithAirVolume/Room with Air Volume  roomWid=1.524 % Parameterized on : 13-Jun-2026 10:47:11  roomHgt=3.048 % Parameterized on : 13-Jun-2026 10:47:11  roomLen=2.4384 % Parameterized on : 13-Jun-2026 10:47:11  htc=30 % Parameterized on : 13-Jun-2026 10:47:16  iniT=300 % Parameterized on : 13-Jun-2026 10:47:16  indxS=14
  Room_A3R1_LivingRoom_C : RoomWithAirVolume/Room with Air Volume  roomWid=4.572 % Parameterized on : 13-Jun-2026 10:47:11  roomHgt=3.048 % Parameterized on : 13-Jun-2026 10:47:11  roomLen=2.4384 % Parameterized on : 13-Jun-2026 10:47:11  htc=30 % Parameterized on : 13-Jun-2026 10:47:16  iniT=300 % Parameterized on : 13-Jun-2026 10:47:16  indxS=15
  Room_A3R2_Bedroom_C : RoomWithAirVolume/Room with Air Volume  roomWid=4.572 % Parameterized on : 13-Jun-2026 10:47:11  roomHgt=3.048 % Parameterized on : 13-Jun-2026 10:47:11  roomLen=4.2672 % Parameterized on : 13-Jun-2026 10:47:11  htc=30 % Parameterized on : 13-Jun-2026 10:47:16  iniT=300 % Parameterized on : 13-Jun-2026 10:47:16  indxS=16
  Room_A3R3_Kitchen_C : RoomWithAirVolume/Room with Air Volume  roomWid=3.9624 % Parameterized on : 13-Jun-2026 10:47:11  roomHgt=3.048 % Parameterized on : 13-Jun-2026 10:47:11  roomLen=2.7432 % Parameterized on : 13-Jun-2026 10:47:11  htc=30 % Parameterized on : 13-Jun-2026 10:47:16  iniT=300 % Parameterized on : 13-Jun-2026 10:47:16  indxS=17
  Room_A3R4_Bathroom_C : RoomWithAirVolume/Room with Air Volume  roomWid=3.6576 % Parameterized on : 13-Jun-2026 10:47:11  roomHgt=3.048 % Parameterized on : 13-Jun-2026 10:47:11  roomLen=2.4384 % Parameterized on : 13-Jun-2026 10:47:11  htc=30 % Parameterized on : 13-Jun-2026 10:47:16  iniT=300 % Parameterized on : 13-Jun-2026 10:47:16  indxS=18
  Room_A3R5_FireExit_C : RoomWithAirVolume/Room with Air Volume  roomWid=2.1336 % Parameterized on : 13-Jun-2026 10:47:11  roomHgt=3.048 % Parameterized on : 13-Jun-2026 10:47:11  roomLen=1.8288 % Parameterized on : 13-Jun-2026 10:47:11  htc=30 % Parameterized on : 13-Jun-2026 10:47:16  iniT=300 % Parameterized on : 13-Jun-2026 10:47:16  indxS=19
  Room_A3R6_Lobby1_C : RoomWithAirVolume/Room with Air Volume  roomWid=2.4384 % Parameterized on : 13-Jun-2026 10:47:11  roomHgt=3.048 % Parameterized on : 13-Jun-2026 10:47:11  roomLen=2.4384 % Parameterized on : 13-Jun-2026 10:47:11  htc=30 % Parameterized on : 13-Jun-2026 10:47:16  iniT=300 % Parameterized on : 13-Jun-2026 10:47:16  indxS=20
  Room_A3R7_Lobby2_C : RoomWithAirVolume/Room with Air Volume  roomWid=1.524 % Parameterized on : 13-Jun-2026 10:47:11  roomHgt=3.048 % Parameterized on : 13-Jun-2026 10:47:11  roomLen=2.4384 % Parameterized on : 13-Jun-2026 10:47:11  htc=30 % Parameterized on : 13-Jun-2026 10:47:16  iniT=300 % Parameterized on : 13-Jun-2026 10:47:16  indxS=21
  Room_A4R1_LivingRoom_D : RoomWithAirVolume/Room with Air Volume  roomWid=4.572 % Parameterized on : 13-Jun-2026 10:47:11  roomHgt=3.048 % Parameterized on : 13-Jun-2026 10:47:11  roomLen=2.4384 % Parameterized on : 13-Jun-2026 10:47:11  htc=30 % Parameterized on : 13-Jun-2026 10:47:16  iniT=300 % Parameterized on : 13-Jun-2026 10:47:16  indxS=22
  Room_A4R2_Bedroom_D : RoomWithAirVolume/Room with Air Volume  roomWid=4.572 % Parameterized on : 13-Jun-2026 10:47:11  roomHgt=3.048 % Parameterized on : 13-Jun-2026 10:47:11  roomLen=4.2672 % Parameterized on : 13-Jun-2026 10:47:11  htc=30 % Parameterized on : 13-Jun-2026 10:47:16  iniT=300 % Parameterized on : 13-Jun-2026 10:47:16  indxS=23
  Room_A4R3_Kitchen_D : RoomWithAirVolume/Room with Air Volume  roomWid=3.9624 % Parameterized on : 13-Jun-2026 10:47:11  roomHgt=3.048 % Parameterized on : 13-Jun-2026 10:47:11  roomLen=2.7432 % Parameterized on : 13-Jun-2026 10:47:11  htc=30 % Parameterized on : 13-Jun-2026 10:47:16  iniT=300 % Parameterized on : 13-Jun-2026 10:47:16  indxS=24
  Room_A4R4_Bathroom_D : RoomWithAirVolume/Room with Air Volume  roomWid=3.6576 % Parameterized on : 13-Jun-2026 10:47:11  roomHgt=3.048 % Parameterized on : 13-Jun-2026 10:47:11  roomLen=2.4384 % Parameterized on : 13-Jun-2026 10:47:11  htc=30 % Parameterized on : 13-Jun-2026 10:47:16  iniT=300 % Parameterized on : 13-Jun-2026 10:47:16  indxS=25
  Room_A4R5_FireExit_D : RoomWithAirVolume/Room with Air Volume  roomWid=2.1336 % Parameterized on : 13-Jun-2026 10:47:11  roomHgt=3.048 % Parameterized on : 13-Jun-2026 10:47:11  roomLen=1.8288 % Parameterized on : 13-Jun-2026 10:47:11  htc=30 % Parameterized on : 13-Jun-2026 10:47:16  iniT=300 % Parameterized on : 13-Jun-2026 10:47:16  indxS=26
  Room_A4R6_Lobby1_D : RoomWithAirVolume/Room with Air Volume  roomWid=2.4384 % Parameterized on : 13-Jun-2026 10:47:11  roomHgt=3.048 % Parameterized on : 13-Jun-2026 10:47:11  roomLen=2.4384 % Parameterized on : 13-Jun-2026 10:47:11  htc=30 % Parameterized on : 13-Jun-2026 10:47:16  iniT=300 % Parameterized on : 13-Jun-2026 10:47:16  indxS=27
  Room_A4R7_Lobby2_D : RoomWithAirVolume/Room with Air Volume  roomWid=1.524 % Parameterized on : 13-Jun-2026 10:47:11  roomHgt=3.048 % Parameterized on : 13-Jun-2026 10:47:11  roomLen=2.4384 % Parameterized on : 13-Jun-2026 10:47:11  htc=30 % Parameterized on : 13-Jun-2026 10:47:16  iniT=300 % Parameterized on : 13-Jun-2026 10:47:16  indxS=28
  Top1 : ConnectionLabel  Label=Top1
  Top10 : ConnectionLabel  Label=Top10
  Top10Lib : ConnectionLabel  Label=Top10
  Top11 : ConnectionLabel  Label=Top11
  Top11Lib : ConnectionLabel  Label=Top11
  Top12 : ConnectionLabel  Label=Top12
  Top12Lib : ConnectionLabel  Label=Top12
  Top13 : ConnectionLabel  Label=Top13
  Top13Lib : ConnectionLabel  Label=Top13
  Top14 : ConnectionLabel  Label=Top14
  Top14Lib : ConnectionLabel  Label=Top14
  Top15 : ConnectionLabel  Label=Top15
  Top15Lib : ConnectionLabel  Label=Top15
  Top16 : ConnectionLabel  Label=Top16
  Top16Lib : ConnectionLabel  Label=Top16
  Top17 : ConnectionLabel  Label=Top17
  Top17Lib : ConnectionLabel  Label=Top17
  Top18 : ConnectionLabel  Label=Top18
  Top18Lib : ConnectionLabel  Label=Top18
  Top19 : ConnectionLabel  Label=Top19
  Top19Lib : ConnectionLabel  Label=Top19
  Top1Lib : ConnectionLabel  Label=Top1
  Top2 : ConnectionLabel  Label=Top2
  Top20 : ConnectionLabel  Label=Top20
  Top20Lib : ConnectionLabel  Label=Top20
  Top21 : ConnectionLabel  Label=Top21
  Top21Lib : ConnectionLabel  Label=Top21
  Top22 : ConnectionLabel  Label=Top22
  Top22Lib : ConnectionLabel  Label=Top22
  Top23 : ConnectionLabel  Label=Top23
  Top23Lib : ConnectionLabel  Label=Top23
  Top24 : ConnectionLabel  Label=Top24
  Top24Lib : ConnectionLabel  Label=Top24
  Top25 : ConnectionLabel  Label=Top25
  Top25Lib : ConnectionLabel  Label=Top25
  Top26 : ConnectionLabel  Label=Top26
  Top26Lib : ConnectionLabel  Label=Top26
  Top27 : ConnectionLabel  Label=Top27
  Top27Lib : ConnectionLabel  Label=Top27
  Top28 : ConnectionLabel  Label=Top28
  Top28Lib : ConnectionLabel  Label=Top28
  Top2Lib : ConnectionLabel  Label=Top2
  Top3 : ConnectionLabel  Label=Top3
  Top3Lib : ConnectionLabel  Label=Top3
  Top4 : ConnectionLabel  Label=Top4
  Top4Lib : ConnectionLabel  Label=Top4
  Top5 : ConnectionLabel  Label=Top5
  Top5Lib : ConnectionLabel  Label=Top5
  Top6 : ConnectionLabel  Label=Top6
  Top6Lib : ConnectionLabel  Label=Top6
  Top7 : ConnectionLabel  Label=Top7
  Top7Lib : ConnectionLabel  Label=Top7
  Top8 : ConnectionLabel  Label=Top8
  Top8Lib : ConnectionLabel  Label=Top8
  Top9 : ConnectionLabel  Label=Top9
  Top9Lib : ConnectionLabel  Label=Top9
  W_A1R1_A1R2 : WallSelector_lib/Wall Selector  optWall=wallModelOption.wallOnly  wallLength=0.00046 % Parameterized on : 13-Jun-2026 10:47:14 m  wallHeight=3.048 % Parameterized on : 13-Jun-2026 10:47:14 m  wallThickness=0.04 % Parameterized on : 13-Jun-2026 10:47:14 m  wallMaterialDen=650 % Parameterized on : 13-Jun-2026 10:47:24 kg/m^3  wallMaterialCp=1100 % Parameterized on : 13-Jun-2026 10:47:24 J/(K*kg)  wallAbsorptivity=0.5  wallThermalK=1.4 % Parameterized on : 13-Jun-2026 10:47:24 W/(K*m)  winLength=1 m  winHeight=0.5 m  winThickness=0.007 m  winMaterialDen=2500 kg/m^3  winMaterialCp=787 J/(K*kg)  winAbsorptivity=0.35  winThermalK=1 W/(K*m)  winTransmissivity=0.45  ventLength=0.1 m  ventHeight=0.1 m  extToWallHTC=30 % Parameterized on : 13-Jun-2026 10:47:24 W/(K*m^2)  intToRoomHTC=30 % Parameterized on : 13-Jun-2026 10:47:24 W/(K*m^2)  iniT=300 % Parameterized on : 13-Jun-2026 10:47:24 K
  W_A1R1_A1R3 : WallSelector_lib/Wall Selector  optWall=wallModelOption.wallOnly  wallLength=3.9624 % Parameterized on : 13-Jun-2026 10:47:14 m  wallHeight=3.048 % Parameterized on : 13-Jun-2026 10:47:14 m  wallThickness=0.04 % Parameterized on : 13-Jun-2026 10:47:14 m  wallMaterialDen=650 % Parameterized on : 13-Jun-2026 10:47:24 kg/m^3  wallMaterialCp=1100 % Parameterized on : 13-Jun-2026 10:47:24 J/(K*kg)  wallAbsorptivity=0.5  wallThermalK=1.4 % Parameterized on : 13-Jun-2026 10:47:24 W/(K*m)  winLength=1 m  winHeight=0.5 m  winThickness=0.007 m  winMaterialDen=2500 kg/m^3  winMaterialCp=787 J/(K*kg)  winAbsorptivity=0.35  winThermalK=1 W/(K*m)  winTransmissivity=0.45  ventLength=0.1 m  ventHeight=0.1 m  extToWallHTC=30 % Parameterized on : 13-Jun-2026 10:47:24 W/(K*m^2)  intToRoomHTC=30 % Parameterized on : 13-Jun-2026 10:47:24 W/(K*m^2)  iniT=300 % Parameterized on : 13-Jun-2026 10:47:24 K
  W_A1R1_A1R4 : WallSelector_lib/Wall Selector  optWall=wallModelOption.wallOnly  wallLength=3.6576 % Parameterized on : 13-Jun-2026 10:47:14 m  wallHeight=3.048 % Parameterized on : 13-Jun-2026 10:47:14 m  wallThickness=0.04 % Parameterized on : 13-Jun-2026 10:47:14 m  wallMaterialDen=650 % Parameterized on : 13-Jun-2026 10:47:24 kg/m^3  wallMaterialCp=1100 % Parameterized on : 13-Jun-2026 10:47:24 J/(K*kg)  wallAbsorptivity=0.5  wallThermalK=1.4 % Parameterized on : 13-Jun-2026 10:47:24 W/(K*m)  winLength=1 m  winHeight=0.5 m  winThickness=0.007 m  winMaterialDen=2500 kg/m^3  winMaterialCp=787 J/(K*kg)  winAbsorptivity=0.35  winThermalK=1 W/(K*m)  winTransmissivity=0.45  ventLength=0.1 m  ventHeight=0.1 m  extToWallHTC=30 % Parameterized on : 13-Jun-2026 10:47:24 W/(K*m^2)  intToRoomHTC=30 % Parameterized on : 13-Jun-2026 10:47:24 W/(K*m^2)  iniT=300 % Parameterized on : 13-Jun-2026 10:47:24 K
  W_A1R1_A1R5 : WallSelector_lib/Wall Selector  optWall=wallModelOption.wallOnly  wallLength=0.6096 % Parameterized on : 13-Jun-2026 10:47:14 m  wallHeight=3.048 % Parameterized on : 13-Jun-2026 10:47:14 m  wallThickness=0.04 % Parameterized on : 13-Jun-2026 10:47:14 m  wallMaterialDen=650 % Parameterized on : 13-Jun-2026 10:47:24 kg/m^3  wallMaterialCp=1100 % Parameterized on : 13-Jun-2026 10:47:24 J/(K*kg)  wallAbsorptivity=0.5  wallThermalK=1.4 % Parameterized on : 13-Jun-2026 10:47:24 W/(K*m)  winLength=1 m  winHeight=0.5 m  winThickness=0.007 m  winMaterialDen=2500 kg/m^3  winMaterialCp=787 J/(K*kg)  winAbsorptivity=0.35  winThermalK=1 W/(K*m)  winTransmissivity=0.45  ventLength=0.1 m  ventHeight=0.1 m  extToWallHTC=30 % Parameterized on : 13-Jun-2026 10:47:24 W/(K*m^2)  intToRoomHTC=30 % Parameterized on : 13-Jun-2026 10:47:24 W/(K*m^2)  iniT=300 % Parameterized on : 13-Jun-2026 10:47:24 K
  W_A1R1_A1R6 : WallSelector_lib/Wall Selector  optWall=wallModelOption.wallOnly  wallLength=0.9144 % Parameterized on : 13-Jun-2026 10:47:14 m  wallHeight=3.048 % Parameterized on : 13-Jun-2026 10:47:14 m  wallThickness=0.04 % Parameterized on : 13-Jun-2026 10:47:14 m  wallMaterialDen=650 % Parameterized on : 13-Jun-2026 10:47:24 kg/m^3  wallMaterialCp=1100 % Parameterized on : 13-Jun-2026 10:47:24 J/(K*kg)  wallAbsorptivity=0.5  wallThermalK=1.4 % Parameterized on : 13-Jun-2026 10:47:24 W/(K*m)  winLength=1 m  winHeight=0.5 m  winThickness=0.007 m  winMaterialDen=2500 kg/m^3  winMaterialCp=787 J/(K*kg)  winAbsorptivity=0.35  winThermalK=1 W/(K*m)  winTransmissivity=0.45  ventLength=0.1 m  ventHeight=0.1 m  extToWallHTC=30 % Parameterized on : 13-Jun-2026 10:47:24 W/(K*m^2)  intToRoomHTC=30 % Parameterized on : 13-Jun-2026 10:47:24 W/(K*m^2)  iniT=300 % Parameterized on : 13-Jun-2026 10:47:24 K
  W_A1R1_A1R7 : WallSelector_lib/Wall Selector  optWall=wallModelOption.wallOnly  wallLength=0.0004572 % Parameterized on : 13-Jun-2026 10:47:14 m  wallHeight=3.048 % Parameterized on : 13-Jun-2026 10:47:14 m  wallThickness=0.04 % Parameterized on : 13-Jun-2026 10:47:14 m  wallMaterialDen=650 % Parameterized on : 13-Jun-2026 10:47:24 kg/m^3  wallMaterialCp=1100 % Parameterized on : 13-Jun-2026 10:47:24 J/(K*kg)  wallAbsorptivity=0.5  wallThermalK=1.4 % Parameterized on : 13-Jun-2026 10:47:24 W/(K*m)  winLength=1 m  winHeight=0.5 m  winThickness=0.007 m  winMaterialDen=2500 kg/m^3  winMaterialCp=787 J/(K*kg)  winAbsorptivity=0.35  winThermalK=1 W/(K*m)  winTransmissivity=0.45  ventLength=0.1 m  ventHeight=0.1 m  extToWallHTC=30 % Parameterized on : 13-Jun-2026 10:47:24 W/(K*m^2)  intToRoomHTC=30 % Parameterized on : 13-Jun-2026 10:47:24 W/(K*m^2)  iniT=300 % Parameterized on : 13-Jun-2026 10:47:24 K
  W_A1R2_A1R3 : WallSelector_lib/Wall Selector  optWall=wallModelOption.wallOnly  wallLength=0.00046 % Parameterized on : 13-Jun-2026 10:47:14 m  wallHeight=3.048 % Parameterized on : 13-Jun-2026 10:47:14 m  wallThickness=0.04 % Parameterized on : 13-Jun-2026 10:47:14 m  wallMaterialDen=650 % Parameterized on : 13-Jun-2026 10:47:24 kg/m^3  wallMaterialCp=1100 % Parameterized on : 13-Jun-2026 10:47:24 J/(K*kg)  wallAbsorptivity=0.5  wallThermalK=1.4 % Parameterized on : 13-Jun-2026 10:47:24 W/(K*m)  winLength=1 m  winHeight=0.5 m  winThickness=0.007 m  winMaterialDen=2500 kg/m^3  winMaterialCp=787 J/(K*kg)  winAbsorptivity=0.35  winThermalK=1 W/(K*m)  winTransmissivity=0.45  ventLength=0.1 m  ventHeight=0.1 m  extToWallHTC=30 % Parameterized on : 13-Jun-2026 10:47:24 W/(K*m^2)  intToRoomHTC=30 % Parameterized on : 13-Jun-2026 10:47:24 W/(K*m^2)  iniT=300 % Parameterized on : 13-Jun-2026 10:47:24 K
  W_A1R2_A1R4 : WallSelector_lib/Wall Selector  optWall=wallModelOption.wallOnly  wallLength=0.00046 % Parameterized on : 13-Jun-2026 10:47:14 m  wallHeight=3.048 % Parameterized on : 13-Jun-2026 10:47:14 m  wallThickness=0.04 % Parameterized on : 13-Jun-2026 10:47:14 m  wallMaterialDen=650 % Parameterized on : 13-Jun-2026 10:47:24 kg/m^3  wallMaterialCp=1100 % Parameterized on : 13-Jun-2026 10:47:24 J/(K*kg)  wallAbsorptivity=0.5  wallThermalK=1.4 % Parameterized on : 13-Jun-2026 10:47:24 W/(K*m)  winLength=1 m  winHeight=0.5 m  winThickness=0.007 m  winMaterialDen=2500 kg/m^3  winMaterialCp=787 J/(K*kg)  winAbsorptivity=0.35  winThermalK=1 W/(K*m)  winTransmissivity=0.45  ventLength=0.1 m  ventHeight=0.1 m  extToWallHTC=30 % Parameterized on : 13-Jun-2026 10:47:24 W/(K*m^2)  intToRoomHTC=30 % Parameterized on : 13-Jun-2026 10:47:24 W/(K*m^2)  iniT=300 % Parameterized on : 13-Jun-2026 10:47:24 K
  W_A1R3_A1R5 : WallSelector_lib/Wall Selector  optWall=wallModelOption.wallOnly  wallLength=0.000396 % Parameterized on : 13-Jun-2026 10:47:14 m  wallHeight=3.048 % Parameterized on : 13-Jun-2026 10:47:14 m  wallThickness=0.04 % Parameterized on : 13-Jun-2026 10:47:14 m  wallMaterialDen=650 % Parameterized on : 13-Jun-2026 10:47:24 kg/m^3  wallMaterialCp=1100 % Parameterized on : 13-Jun-2026 10:47:24 J/(K*kg)  wallAbsorptivity=0.5  wallThermalK=1.4 % Parameterized on : 13-Jun-2026 10:47:24 W/(K*m)  winLength=1 m  winHeight=0.5 m  winThickness=0.007 m  winMaterialDen=2500 kg/m^3  winMaterialCp=787 J/(K*kg)  winAbsorptivity=0.35  winThermalK=1 W/(K*m)  winTransmissivity=0.45  ventLength=0.1 m  ventHeight=0.1 m  extToWallHTC=30 % Parameterized on : 13-Jun-2026 10:47:24 W/(K*m^2)  intToRoomHTC=30 % Parameterized on : 13-Jun-2026 10:47:24 W/(K*m^2)  iniT=300 % Parameterized on : 13-Jun-2026 10:47:24 K
  W_A1R4_A1R6 : WallSelector_lib/Wall Selector  optWall=wallModelOption.wallOnly  wallLength=0.000366 % Parameterized on : 13-Jun-2026 10:47:14 m  wallHeight=3.048 % Parameterized on : 13-Jun-2026 10:47:14 m  wallThickness=0.04 % Parameterized on : 13-Jun-2026 10:47:14 m  wallMaterialDen=650 % Parameterized on : 13-Jun-2026 10:47:24 kg/m^3  wallMaterialCp=1100 % Parameterized on : 13-Jun-2026 10:47:24 J/(K*kg)  wallAbsorptivity=0.5  wallThermalK=1.4 % Parameterized on : 13-Jun-2026 10:47:24 W/(K*m)  winLength=1 m  winHeight=0.5 m  winThickness=0.007 m  winMaterialDen=2500 kg/m^3  winMaterialCp=787 J/(K*kg)  winAbsorptivity=0.35  winThermalK=1 W/(K*m)  winTransmissivity=0.45  ventLength=0.1 m  ventHeight=0.1 m  extToWallHTC=30 % Parameterized on : 13-Jun-2026 10:47:24 W/(K*m^2)  intToRoomHTC=30 % Parameterized on : 13-Jun-2026 10:47:24 W/(K*m^2)  iniT=300 % Parameterized on : 13-Jun-2026 10:47:24 K
  W_A1R5_A1R7 : WallSelector_lib/Wall Selector  optWall=wallModelOption.wallOnly  wallLength=1.524 % Parameterized on : 13-Jun-2026 10:47:14 m  wallHeight=3.048 % Parameterized on : 13-Jun-2026 10:47:14 m  wallThickness=0.04 % Parameterized on : 13-Jun-2026 10:47:14 m  wallMaterialDen=650 % Parameterized on : 13-Jun-2026 10:47:24 kg/m^3  wallMaterialCp=1100 % Parameterized on : 13-Jun-2026 10:47:24 J/(K*kg)  wallAbsorptivity=0.5  wallThermalK=1.4 % Parameterized on : 13-Jun-2026 10:47:24 W/(K*m)  winLength=1 m  winHeight=0.5 m  winThickness=0.007 m  winMaterialDen=2500 kg/m^3  winMaterialCp=787 J/(K*kg)  winAbsorptivity=0.35  winThermalK=1 W/(K*m)  winTransmissivity=0.45  ventLength=0.1 m  ventHeight=0.1 m  extToWallHTC=30 % Parameterized on : 13-Jun-2026 10:47:24 W/(K*m^2)  intToRoomHTC=30 % Parameterized on : 13-Jun-2026 10:47:24 W/(K*m^2)  iniT=300 % Parameterized on : 13-Jun-2026 10:47:24 K
  W_A1R6_A1R7 : WallSelector_lib/Wall Selector  optWall=wallModelOption.wallOnly  wallLength=1.524 % Parameterized on : 13-Jun-2026 10:47:14 m  wallHeight=3.048 % Parameterized on : 13-Jun-2026 10:47:14 m  wallThickness=0.04 % Parameterized on : 13-Jun-2026 10:47:14 m  wallMaterialDen=650 % Parameterized on : 13-Jun-2026 10:47:24 kg/m^3  wallMaterialCp=1100 % Parameterized on : 13-Jun-2026 10:47:24 J/(K*kg)  wallAbsorptivity=0.5  wallThermalK=1.4 % Parameterized on : 13-Jun-2026 10:47:24 W/(K*m)  winLength=1 m  winHeight=0.5 m  winThickness=0.007 m  winMaterialDen=2500 kg/m^3  winMaterialCp=787 J/(K*kg)  winAbsorptivity=0.35  winThermalK=1 W/(K*m)  winTransmissivity=0.45  ventLength=0.1 m  ventHeight=0.1 m  extToWallHTC=30 % Parameterized on : 13-Jun-2026 10:47:24 W/(K*m^2)  intToRoomHTC=30 % Parameterized on : 13-Jun-2026 10:47:24 W/(K*m^2)  iniT=300 % Parameterized on : 13-Jun-2026 10:47:25 K
  W_A2R1_A2R2 : WallSelector_lib/Wall Selector  optWall=wallModelOption.wallOnly  wallLength=0.00046 % Parameterized on : 13-Jun-2026 10:47:14 m  wallHeight=3.048 % Parameterized on : 13-Jun-2026 10:47:14 m  wallThickness=0.04 % Parameterized on : 13-Jun-2026 10:47:14 m  wallMaterialDen=650 % Parameterized on : 13-Jun-2026 10:47:25 kg/m^3  wallMaterialCp=1100 % Parameterized on : 13-Jun-2026 10:47:25 J/(K*kg)  wallAbsorptivity=0.5  wallThermalK=1.4 % Parameterized on : 13-Jun-2026 10:47:25 W/(K*m)  winLength=1 m  winHeight=0.5 m  winThickness=0.007 m  winMaterialDen=2500 kg/m^3  winMaterialCp=787 J/(K*kg)  winAbsorptivity=0.35  winThermalK=1 W/(K*m)  winTransmissivity=0.45  ventLength=0.1 m  ventHeight=0.1 m  extToWallHTC=30 % Parameterized on : 13-Jun-2026 10:47:25 W/(K*m^2)  intToRoomHTC=30 % Parameterized on : 13-Jun-2026 10:47:25 W/(K*m^2)  iniT=300 % Parameterized on : 13-Jun-2026 10:47:25 K
  W_A2R1_A2R3 : WallSelector_lib/Wall Selector  optWall=wallModelOption.wallOnly  wallLength=3.9624 % Parameterized on : 13-Jun-2026 10:47:14 m  wallHeight=3.048 % Parameterized on : 13-Jun-2026 10:47:14 m  wallThickness=0.04 % Parameterized on : 13-Jun-2026 10:47:14 m  wallMaterialDen=650 % Parameterized on : 13-Jun-2026 10:47:25 kg/m^3  wallMaterialCp=1100 % Parameterized on : 13-Jun-2026 10:47:25 J/(K*kg)  wallAbsorptivity=0.5  wallThermalK=1.4 % Parameterized on : 13-Jun-2026 10:47:25 W/(K*m)  winLength=1 m  winHeight=0.5 m  winThickness=0.007 m  winMaterialDen=2500 kg/m^3  winMaterialCp=787 J/(K*kg)  winAbsorptivity=0.35  winThermalK=1 W/(K*m)  winTransmissivity=0.45  ventLength=0.1 m  ventHeight=0.1 m  extToWallHTC=30 % Parameterized on : 13-Jun-2026 10:47:25 W/(K*m^2)  intToRoomHTC=30 % Parameterized on : 13-Jun-2026 10:47:25 W/(K*m^2)  iniT=300 % Parameterized on : 13-Jun-2026 10:47:25 K
  W_A2R1_A2R4 : WallSelector_lib/Wall Selector  optWall=wallModelOption.wallOnly  wallLength=3.6576 % Parameterized on : 13-Jun-2026 10:47:14 m  wallHeight=3.048 % Parameterized on : 13-Jun-2026 10:47:14 m  wallThickness=0.04 % Parameterized on : 13-Jun-2026 10:47:14 m  wallMaterialDen=650 % Parameterized on : 13-Jun-2026 10:47:25 kg/m^3  wallMaterialCp=1100 % Parameterized on : 13-Jun-2026 10:47:25 J/(K*kg)  wallAbsorptivity=0.5  wallThermalK=1.4 % Parameterized on : 13-Jun-2026 10:47:25 W/(K*m)  winLength=1 m  winHeight=0.5 m  winThickness=0.007 m  winMaterialDen=2500 kg/m^3  winMaterialCp=787 J/(K*kg)  winAbsorptivity=0.35  winThermalK=1 W/(K*m)  winTransmissivity=0.45  ventLength=0.1 m  ventHeight=0.1 m  extToWallHTC=30 % Parameterized on : 13-Jun-2026 10:47:25 W/(K*m^2)  intToRoomHTC=30 % Parameterized on : 13-Jun-2026 10:47:25 W/(K*m^2)  iniT=300 % Parameterized on : 13-Jun-2026 10:47:25 K
  W_A2R1_A2R5 : WallSelector_lib/Wall Selector  optWall=wallModelOption.wallOnly  wallLength=0.6096 % Parameterized on : 13-Jun-2026 10:47:14 m  wallHeight=3.048 % Parameterized on : 13-Jun-2026 10:47:14 m  wallThickness=0.04 % Parameterized on : 13-Jun-2026 10:47:14 m  wallMaterialDen=650 % Parameterized on : 13-Jun-2026 10:47:25 kg/m^3  wallMaterialCp=1100 % Parameterized on : 13-Jun-2026 10:47:25 J/(K*kg)  wallAbsorptivity=0.5  wallThermalK=1.4 % Parameterized on : 13-Jun-2026 10:47:25 W/(K*m)  winLength=1 m  winHeight=0.5 m  winThickness=0.007 m  winMaterialDen=2500 kg/m^3  winMaterialCp=787 J/(K*kg)  winAbsorptivity=0.35  winThermalK=1 W/(K*m)  winTransmissivity=0.45  ventLength=0.1 m  ventHeight=0.1 m  extToWallHTC=30 % Parameterized on : 13-Jun-2026 10:47:25 W/(K*m^2)  intToRoomHTC=30 % Parameterized on : 13-Jun-2026 10:47:25 W/(K*m^2)  iniT=300 % Parameterized on : 13-Jun-2026 10:47:25 K
  W_A2R1_A2R6 : WallSelector_lib/Wall Selector  optWall=wallModelOption.wallOnly  wallLength=0.9144 % Parameterized on : 13-Jun-2026 10:47:14 m  wallHeight=3.048 % Parameterized on : 13-Jun-2026 10:47:14 m  wallThickness=0.04 % Parameterized on : 13-Jun-2026 10:47:14 m  wallMaterialDen=650 % Parameterized on : 13-Jun-2026 10:47:25 kg/m^3  wallMaterialCp=1100 % Parameterized on : 13-Jun-2026 10:47:25 J/(K*kg)  wallAbsorptivity=0.5  wallThermalK=1.4 % Parameterized on : 13-Jun-2026 10:47:25 W/(K*m)  winLength=1 m  winHeight=0.5 m  winThickness=0.007 m  winMaterialDen=2500 kg/m^3  winMaterialCp=787 J/(K*kg)  winAbsorptivity=0.35  winThermalK=1 W/(K*m)  winTransmissivity=0.45  ventLength=0.1 m  ventHeight=0.1 m  extToWallHTC=30 % Parameterized on : 13-Jun-2026 10:47:25 W/(K*m^2)  intToRoomHTC=30 % Parameterized on : 13-Jun-2026 10:47:25 W/(K*m^2)  iniT=300 % Parameterized on : 13-Jun-2026 10:47:25 K
  W_A2R1_A2R7 : WallSelector_lib/Wall Selector  optWall=wallModelOption.wallOnly  wallLength=0.00046 % Parameterized on : 13-Jun-2026 10:47:14 m  wallHeight=3.048 % Parameterized on : 13-Jun-2026 10:47:14 m  wallThickness=0.04 % Parameterized on : 13-Jun-2026 10:47:14 m  wallMaterialDen=650 % Parameterized on : 13-Jun-2026 10:47:25 kg/m^3  wallMaterialCp=1100 % Parameterized on : 13-Jun-2026 10:47:25 J/(K*kg)  wallAbsorptivity=0.5  wallThermalK=1.4 % Parameterized on : 13-Jun-2026 10:47:25 W/(K*m)  winLength=1 m  winHeight=0.5 m  winThickness=0.007 m  winMaterialDen=2500 kg/m^3  winMaterialCp=787 J/(K*kg)  winAbsorptivity=0.35  winThermalK=1 W/(K*m)  winTransmissivity=0.45  ventLength=0.1 m  ventHeight=0.1 m  extToWallHTC=30 % Parameterized on : 13-Jun-2026 10:47:25 W/(K*m^2)  intToRoomHTC=30 % Parameterized on : 13-Jun-2026 10:47:25 W/(K*m^2)  iniT=300 % Parameterized on : 13-Jun-2026 10:47:25 K
  W_A2R2_A2R3 : WallSelector_lib/Wall Selector  optWall=wallModelOption.wallOnly  wallLength=0.00046 % Parameterized on : 13-Jun-2026 10:47:14 m  wallHeight=3.048 % Parameterized on : 13-Jun-2026 10:47:14 m  wallThickness=0.04 % Parameterized on : 13-Jun-2026 10:47:14 m  wallMaterialDen=650 % Parameterized on : 13-Jun-2026 10:47:25 kg/m^3  wallMaterialCp=1100 % Parameterized on : 13-Jun-2026 10:47:25 J/(K*kg)  wallAbsorptivity=0.5  wallThermalK=1.4 % Parameterized on : 13-Jun-2026 10:47:25 W/(K*m)  winLength=1 m  winHeight=0.5 m  winThickness=0.007 m  winMaterialDen=2500 kg/m^3  winMaterialCp=787 J/(K*kg)  winAbsorptivity=0.35  winThermalK=1 W/(K*m)  winTransmissivity=0.45  ventLength=0.1 m  ventHeight=0.1 m  extToWallHTC=30 % Parameterized on : 13-Jun-2026 10:47:25 W/(K*m^2)  intToRoomHTC=30 % Parameterized on : 13-Jun-2026 10:47:25 W/(K*m^2)  iniT=300 % Parameterized on : 13-Jun-2026 10:47:25 K
  W_A2R2_A2R4 : WallSelector_lib/Wall Selector  optWall=wallModelOption.wallOnly  wallLength=0.00046 % Parameterized on : 13-Jun-2026 10:47:14 m  wallHeight=3.048 % Parameterized on : 13-Jun-2026 10:47:14 m  wallThickness=0.04 % Parameterized on : 13-Jun-2026 10:47:14 m  wallMaterialDen=650 % Parameterized on : 13-Jun-2026 10:47:25 kg/m^3  wallMaterialCp=1100 % Parameterized on : 13-Jun-2026 10:47:25 J/(K*kg)  wallAbsorptivity=0.5  wallThermalK=1.4 % Parameterized on : 13-Jun-2026 10:47:25 W/(K*m)  winLength=1 m  winHeight=0.5 m  winThickness=0.007 m  winMaterialDen=2500 kg/m^3  winMaterialCp=787 J/(K*kg)  winAbsorptivity=0.35  winThermalK=1 W/(K*m)  winTransmissivity=0.45  ventLength=0.1 m  ventHeight=0.1 m  extToWallHTC=30 % Parameterized on : 13-Jun-2026 10:47:25 W/(K*m^2)  intToRoomHTC=30 % Parameterized on : 13-Jun-2026 10:47:25 W/(K*m^2)  iniT=300 % Parameterized on : 13-Jun-2026 10:47:25 K
  W_A2R3_A2R5 : WallSelector_lib/Wall Selector  optWall=wallModelOption.wallOnly  wallLength=0.0004 % Parameterized on : 13-Jun-2026 10:47:14 m  wallHeight=3.048 % Parameterized on : 13-Jun-2026 10:47:14 m  wallThickness=0.04 % Parameterized on : 13-Jun-2026 10:47:14 m  wallMaterialDen=650 % Parameterized on : 13-Jun-2026 10:47:25 kg/m^3  wallMaterialCp=1100 % Parameterized on : 13-Jun-2026 10:47:25 J/(K*kg)  wallAbsorptivity=0.5  wallThermalK=1.4 % Parameterized on : 13-Jun-2026 10:47:25 W/(K*m)  winLength=1 m  winHeight=0.5 m  winThickness=0.007 m  winMaterialDen=2500 kg/m^3  winMaterialCp=787 J/(K*kg)  winAbsorptivity=0.35  winThermalK=1 W/(K*m)  winTransmissivity=0.45  ventLength=0.1 m  ventHeight=0.1 m  extToWallHTC=30 % Parameterized on : 13-Jun-2026 10:47:25 W/(K*m^2)  intToRoomHTC=30 % Parameterized on : 13-Jun-2026 10:47:25 W/(K*m^2)  iniT=300 % Parameterized on : 13-Jun-2026 10:47:25 K
  W_A2R4_A2R6 : WallSelector_lib/Wall Selector  optWall=wallModelOption.wallOnly  wallLength=0.00037 % Parameterized on : 13-Jun-2026 10:47:14 m  wallHeight=3.048 % Parameterized on : 13-Jun-2026 10:47:14 m  wallThickness=0.04 % Parameterized on : 13-Jun-2026 10:47:14 m  wallMaterialDen=650 % Parameterized on : 13-Jun-2026 10:47:25 kg/m^3  wallMaterialCp=1100 % Parameterized on : 13-Jun-2026 10:47:25 J/(K*kg)  wallAbsorptivity=0.5  wallThermalK=1.4 % Parameterized on : 13-Jun-2026 10:47:25 W/(K*m)  winLength=1 m  winHeight=0.5 m  winThickness=0.007 m  winMaterialDen=2500 kg/m^3  winMaterialCp=787 J/(K*kg)  winAbsorptivity=0.35  winThermalK=1 W/(K*m)  winTransmissivity=0.45  ventLength=0.1 m  ventHeight=0.1 m  extToWallHTC=30 % Parameterized on : 13-Jun-2026 10:47:25 W/(K*m^2)  intToRoomHTC=30 % Parameterized on : 13-Jun-2026 10:47:25 W/(K*m^2)  iniT=300 % Parameterized on : 13-Jun-2026 10:47:25 K
  W_A2R5_A2R7 : WallSelector_lib/Wall Selector  optWall=wallModelOption.wallOnly  wallLength=1.524 % Parameterized on : 13-Jun-2026 10:47:14 m  wallHeight=3.048 % Parameterized on : 13-Jun-2026 10:47:14 m  wallThickness=0.04 % Parameterized on : 13-Jun-2026 10:47:14 m  wallMaterialDen=650 % Parameterized on : 13-Jun-2026 10:47:25 kg/m^3  wallMaterialCp=1100 % Parameterized on : 13-Jun-2026 10:47:25 J/(K*kg)  wallAbsorptivity=0.5  wallThermalK=1.4 % Parameterized on : 13-Jun-2026 10:47:25 W/(K*m)  winLength=1 m  winHeight=0.5 m  winThickness=0.007 m  winMaterialDen=2500 kg/m^3  winMaterialCp=787 J/(K*kg)  winAbsorptivity=0.35  winThermalK=1 W/(K*m)  winTransmissivity=0.45  ventLength=0.1 m  ventHeight=0.1 m  extToWallHTC=30 % Parameterized on : 13-Jun-2026 10:47:25 W/(K*m^2)  intToRoomHTC=30 % Parameterized on : 13-Jun-2026 10:47:25 W/(K*m^2)  iniT=300 % Parameterized on : 13-Jun-2026 10:47:25 K
  W_A2R6_A2R7 : WallSelector_lib/Wall Selector  optWall=wallModelOption.wallOnly  wallLength=1.524 % Parameterized on : 13-Jun-2026 10:47:14 m  wallHeight=3.048 % Parameterized on : 13-Jun-2026 10:47:14 m  wallThickness=0.04 % Parameterized on : 13-Jun-2026 10:47:14 m  wallMaterialDen=650 % Parameterized on : 13-Jun-2026 10:47:25 kg/m^3  wallMaterialCp=1100 % Parameterized on : 13-Jun-2026 10:47:25 J/(K*kg)  wallAbsorptivity=0.5  wallThermalK=1.4 % Parameterized on : 13-Jun-2026 10:47:25 W/(K*m)  winLength=1 m  winHeight=0.5 m  winThickness=0.007 m  winMaterialDen=2500 kg/m^3  winMaterialCp=787 J/(K*kg)  winAbsorptivity=0.35  winThermalK=1 W/(K*m)  winTransmissivity=0.45  ventLength=0.1 m  ventHeight=0.1 m  extToWallHTC=30 % Parameterized on : 13-Jun-2026 10:47:25 W/(K*m^2)  intToRoomHTC=30 % Parameterized on : 13-Jun-2026 10:47:25 W/(K*m^2)  iniT=300 % Parameterized on : 13-Jun-2026 10:47:25 K
  W_A3R1_A3R2 : WallSelector_lib/Wall Selector  optWall=wallModelOption.wallOnly  wallLength=0.00046 % Parameterized on : 13-Jun-2026 10:47:14 m  wallHeight=3.048 % Parameterized on : 13-Jun-2026 10:47:14 m  wallThickness=0.04 % Parameterized on : 13-Jun-2026 10:47:14 m  wallMaterialDen=650 % Parameterized on : 13-Jun-2026 10:47:25 kg/m^3  wallMaterialCp=1100 % Parameterized on : 13-Jun-2026 10:47:25 J/(K*kg)  wallAbsorptivity=0.5  wallThermalK=1.4 % Parameterized on : 13-Jun-2026 10:47:25 W/(K*m)  winLength=1 m  winHeight=0.5 m  winThickness=0.007 m  winMaterialDen=2500 kg/m^3  winMaterialCp=787 J/(K*kg)  winAbsorptivity=0.35  winThermalK=1 W/(K*m)  winTransmissivity=0.45  ventLength=0.1 m  ventHeight=0.1 m  extToWallHTC=30 % Parameterized on : 13-Jun-2026 10:47:25 W/(K*m^2)  intToRoomHTC=30 % Parameterized on : 13-Jun-2026 10:47:25 W/(K*m^2)  iniT=300 % Parameterized on : 13-Jun-2026 10:47:25 K
  W_A3R1_A3R3 : WallSelector_lib/Wall Selector  optWall=wallModelOption.wallOnly  wallLength=3.9624 % Parameterized on : 13-Jun-2026 10:47:14 m  wallHeight=3.048 % Parameterized on : 13-Jun-2026 10:47:14 m  wallThickness=0.04 % Parameterized on : 13-Jun-2026 10:47:14 m  wallMaterialDen=650 % Parameterized on : 13-Jun-2026 10:47:25 kg/m^3  wallMaterialCp=1100 % Parameterized on : 13-Jun-2026 10:47:25 J/(K*kg)  wallAbsorptivity=0.5  wallThermalK=1.4 % Parameterized on : 13-Jun-2026 10:47:25 W/(K*m)  winLength=1 m  winHeight=0.5 m  winThickness=0.007 m  winMaterialDen=2500 kg/m^3  winMaterialCp=787 J/(K*kg)  winAbsorptivity=0.35  winThermalK=1 W/(K*m)  winTransmissivity=0.45  ventLength=0.1 m  ventHeight=0.1 m  extToWallHTC=30 % Parameterized on : 13-Jun-2026 10:47:25 W/(K*m^2)  intToRoomHTC=30 % Parameterized on : 13-Jun-2026 10:47:25 W/(K*m^2)  iniT=300 % Parameterized on : 13-Jun-2026 10:47:25 K
  W_A3R1_A3R4 : WallSelector_lib/Wall Selector  optWall=wallModelOption.wallOnly  wallLength=3.6576 % Parameterized on : 13-Jun-2026 10:47:14 m  wallHeight=3.048 % Parameterized on : 13-Jun-2026 10:47:14 m  wallThickness=0.04 % Parameterized on : 13-Jun-2026 10:47:14 m  wallMaterialDen=650 % Parameterized on : 13-Jun-2026 10:47:25 kg/m^3  wallMaterialCp=1100 % Parameterized on : 13-Jun-2026 10:47:25 J/(K*kg)  wallAbsorptivity=0.5  wallThermalK=1.4 % Parameterized on : 13-Jun-2026 10:47:25 W/(K*m)  winLength=1 m  winHeight=0.5 m  winThickness=0.007 m  winMaterialDen=2500 kg/m^3  winMaterialCp=787 J/(K*kg)  winAbsorptivity=0.35  winThermalK=1 W/(K*m)  winTransmissivity=0.45  ventLength=0.1 m  ventHeight=0.1 m  extToWallHTC=30 % Parameterized on : 13-Jun-2026 10:47:25 W/(K*m^2)  intToRoomHTC=30 % Parameterized on : 13-Jun-2026 10:47:25 W/(K*m^2)  iniT=300 % Parameterized on : 13-Jun-2026 10:47:25 K
  W_A3R1_A3R5 : WallSelector_lib/Wall Selector  optWall=wallModelOption.wallOnly  wallLength=0.6096 % Parameterized on : 13-Jun-2026 10:47:14 m  wallHeight=3.048 % Parameterized on : 13-Jun-2026 10:47:14 m  wallThickness=0.04 % Parameterized on : 13-Jun-2026 10:47:14 m  wallMaterialDen=650 % Parameterized on : 13-Jun-2026 10:47:25 kg/m^3  wallMaterialCp=1100 % Parameterized on : 13-Jun-2026 10:47:25 J/(K*kg)  wallAbsorptivity=0.5  wallThermalK=1.4 % Parameterized on : 13-Jun-2026 10:47:25 W/(K*m)  winLength=1 m  winHeight=0.5 m  winThickness=0.007 m  winMaterialDen=2500 kg/m^3  winMaterialCp=787 J/(K*kg)  winAbsorptivity=0.35  winThermalK=1 W/(K*m)  winTransmissivity=0.45  ventLength=0.1 m  ventHeight=0.1 m  extToWallHTC=30 % Parameterized on : 13-Jun-2026 10:47:25 W/(K*m^2)  intToRoomHTC=30 % Parameterized on : 13-Jun-2026 10:47:25 W/(K*m^2)  iniT=300 % Parameterized on : 13-Jun-2026 10:47:25 K
  W_A3R1_A3R6 : WallSelector_lib/Wall Selector  optWall=wallModelOption.wallOnly  wallLength=0.9144 % Parameterized on : 13-Jun-2026 10:47:14 m  wallHeight=3.048 % Parameterized on : 13-Jun-2026 10:47:14 m  wallThickness=0.04 % Parameterized on : 13-Jun-2026 10:47:14 m  wallMaterialDen=650 % Parameterized on : 13-Jun-2026 10:47:25 kg/m^3  wallMaterialCp=1100 % Parameterized on : 13-Jun-2026 10:47:25 J/(K*kg)  wallAbsorptivity=0.5  wallThermalK=1.4 % Parameterized on : 13-Jun-2026 10:47:25 W/(K*m)  winLength=1 m  winHeight=0.5 m  winThickness=0.007 m  winMaterialDen=2500 kg/m^3  winMaterialCp=787 J/(K*kg)  winAbsorptivity=0.35  winThermalK=1 W/(K*m)  winTransmissivity=0.45  ventLength=0.1 m  ventHeight=0.1 m  extToWallHTC=30 % Parameterized on : 13-Jun-2026 10:47:25 W/(K*m^2)  intToRoomHTC=30 % Parameterized on : 13-Jun-2026 10:47:25 W/(K*m^2)  iniT=300 % Parameterized on : 13-Jun-2026 10:47:25 K
  W_A3R1_A3R7 : WallSelector_lib/Wall Selector  optWall=wallModelOption.wallOnly  wallLength=0.0004572 % Parameterized on : 13-Jun-2026 10:47:14 m  wallHeight=3.048 % Parameterized on : 13-Jun-2026 10:47:14 m  wallThickness=0.04 % Parameterized on : 13-Jun-2026 10:47:14 m  wallMaterialDen=650 % Parameterized on : 13-Jun-2026 10:47:25 kg/m^3  wallMaterialCp=1100 % Parameterized on : 13-Jun-2026 10:47:25 J/(K*kg)  wallAbsorptivity=0.5  wallThermalK=1.4 % Parameterized on : 13-Jun-2026 10:47:25 W/(K*m)  winLength=1 m  winHeight=0.5 m  winThickness=0.007 m  winMaterialDen=2500 kg/m^3  winMaterialCp=787 J/(K*kg)  winAbsorptivity=0.35  winThermalK=1 W/(K*m)  winTransmissivity=0.45  ventLength=0.1 m  ventHeight=0.1 m  extToWallHTC=30 % Parameterized on : 13-Jun-2026 10:47:25 W/(K*m^2)  intToRoomHTC=30 % Parameterized on : 13-Jun-2026 10:47:25 W/(K*m^2)  iniT=300 % Parameterized on : 13-Jun-2026 10:47:25 K
  W_A3R2_A3R3 : WallSelector_lib/Wall Selector  optWall=wallModelOption.wallOnly  wallLength=0.00046 % Parameterized on : 13-Jun-2026 10:47:14 m  wallHeight=3.048 % Parameterized on : 13-Jun-2026 10:47:14 m  wallThickness=0.04 % Parameterized on : 13-Jun-2026 10:47:14 m  wallMaterialDen=650 % Parameterized on : 13-Jun-2026 10:47:25 kg/m^3  wallMaterialCp=1100 % Parameterized on : 13-Jun-2026 10:47:25 J/(K*kg)  wallAbsorptivity=0.5  wallThermalK=1.4 % Parameterized on : 13-Jun-2026 10:47:25 W/(K*m)  winLength=1 m  winHeight=0.5 m  winThickness=0.007 m  winMaterialDen=2500 kg/m^3  winMaterialCp=787 J/(K*kg)  winAbsorptivity=0.35  winThermalK=1 W/(K*m)  winTransmissivity=0.45  ventLength=0.1 m  ventHeight=0.1 m  extToWallHTC=30 % Parameterized on : 13-Jun-2026 10:47:25 W/(K*m^2)  intToRoomHTC=30 % Parameterized on : 13-Jun-2026 10:47:25 W/(K*m^2)  iniT=300 % Parameterized on : 13-Jun-2026 10:47:25 K
  W_A3R2_A3R4 : WallSelector_lib/Wall Selector  optWall=wallModelOption.wallOnly  wallLength=0.00046 % Parameterized on : 13-Jun-2026 10:47:14 m  wallHeight=3.048 % Parameterized on : 13-Jun-2026 10:47:14 m  wallThickness=0.04 % Parameterized on : 13-Jun-2026 10:47:14 m  wallMaterialDen=650 % Parameterized on : 13-Jun-2026 10:47:25 kg/m^3  wallMaterialCp=1100 % Parameterized on : 13-Jun-2026 10:47:25 J/(K*kg)  wallAbsorptivity=0.5  wallThermalK=1.4 % Parameterized on : 13-Jun-2026 10:47:25 W/(K*m)  winLength=1 m  winHeight=0.5 m  winThickness=0.007 m  winMaterialDen=2500 kg/m^3  winMaterialCp=787 J/(K*kg)  winAbsorptivity=0.35  winThermalK=1 W/(K*m)  winTransmissivity=0.45  ventLength=0.1 m  ventHeight=0.1 m  extToWallHTC=30 % Parameterized on : 13-Jun-2026 10:47:25 W/(K*m^2)  intToRoomHTC=30 % Parameterized on : 13-Jun-2026 10:47:25 W/(K*m^2)  iniT=300 % Parameterized on : 13-Jun-2026 10:47:25 K
  W_A3R3_A3R5 : WallSelector_lib/Wall Selector  optWall=wallModelOption.wallOnly  wallLength=0.000396 % Parameterized on : 13-Jun-2026 10:47:14 m  wallHeight=3.048 % Parameterized on : 13-Jun-2026 10:47:14 m  wallThickness=0.04 % Parameterized on : 13-Jun-2026 10:47:14 m  wallMaterialDen=650 % Parameterized on : 13-Jun-2026 10:47:25 kg/m^3  wallMaterialCp=1100 % Parameterized on : 13-Jun-2026 10:47:25 J/(K*kg)  wallAbsorptivity=0.5  wallThermalK=1.4 % Parameterized on : 13-Jun-2026 10:47:25 W/(K*m)  winLength=1 m  winHeight=0.5 m  winThickness=0.007 m  winMaterialDen=2500 kg/m^3  winMaterialCp=787 J/(K*kg)  winAbsorptivity=0.35  winThermalK=1 W/(K*m)  winTransmissivity=0.45  ventLength=0.1 m  ventHeight=0.1 m  extToWallHTC=30 % Parameterized on : 13-Jun-2026 10:47:25 W/(K*m^2)  intToRoomHTC=30 % Parameterized on : 13-Jun-2026 10:47:25 W/(K*m^2)  iniT=300 % Parameterized on : 13-Jun-2026 10:47:25 K
  W_A3R4_A3R6 : WallSelector_lib/Wall Selector  optWall=wallModelOption.wallOnly  wallLength=0.000366 % Parameterized on : 13-Jun-2026 10:47:14 m  wallHeight=3.048 % Parameterized on : 13-Jun-2026 10:47:14 m  wallThickness=0.04 % Parameterized on : 13-Jun-2026 10:47:14 m  wallMaterialDen=650 % Parameterized on : 13-Jun-2026 10:47:25 kg/m^3  wallMaterialCp=1100 % Parameterized on : 13-Jun-2026 10:47:25 J/(K*kg)  wallAbsorptivity=0.5  wallThermalK=1.4 % Parameterized on : 13-Jun-2026 10:47:25 W/(K*m)  winLength=1 m  winHeight=0.5 m  winThickness=0.007 m  winMaterialDen=2500 kg/m^3  winMaterialCp=787 J/(K*kg)  winAbsorptivity=0.35  winThermalK=1 W/(K*m)  winTransmissivity=0.45  ventLength=0.1 m  ventHeight=0.1 m  extToWallHTC=30 % Parameterized on : 13-Jun-2026 10:47:25 W/(K*m^2)  intToRoomHTC=30 % Parameterized on : 13-Jun-2026 10:47:25 W/(K*m^2)  iniT=300 % Parameterized on : 13-Jun-2026 10:47:25 K
  W_A3R5_A3R7 : WallSelector_lib/Wall Selector  optWall=wallModelOption.wallOnly  wallLength=1.524 % Parameterized on : 13-Jun-2026 10:47:14 m  wallHeight=3.048 % Parameterized on : 13-Jun-2026 10:47:14 m  wallThickness=0.04 % Parameterized on : 13-Jun-2026 10:47:14 m  wallMaterialDen=650 % Parameterized on : 13-Jun-2026 10:47:25 kg/m^3  wallMaterialCp=1100 % Parameterized on : 13-Jun-2026 10:47:25 J/(K*kg)  wallAbsorptivity=0.5  wallThermalK=1.4 % Parameterized on : 13-Jun-2026 10:47:25 W/(K*m)  winLength=1 m  winHeight=0.5 m  winThickness=0.007 m  winMaterialDen=2500 kg/m^3  winMaterialCp=787 J/(K*kg)  winAbsorptivity=0.35  winThermalK=1 W/(K*m)  winTransmissivity=0.45  ventLength=0.1 m  ventHeight=0.1 m  extToWallHTC=30 % Parameterized on : 13-Jun-2026 10:47:25 W/(K*m^2)  intToRoomHTC=30 % Parameterized on : 13-Jun-2026 10:47:25 W/(K*m^2)  iniT=300 % Parameterized on : 13-Jun-2026 10:47:25 K
  W_A3R6_A3R7 : WallSelector_lib/Wall Selector  optWall=wallModelOption.wallOnly  wallLength=1.524 % Parameterized on : 13-Jun-2026 10:47:14 m  wallHeight=3.048 % Parameterized on : 13-Jun-2026 10:47:14 m  wallThickness=0.04 % Parameterized on : 13-Jun-2026 10:47:14 m  wallMaterialDen=650 % Parameterized on : 13-Jun-2026 10:47:25 kg/m^3  wallMaterialCp=1100 % Parameterized on : 13-Jun-2026 10:47:25 J/(K*kg)  wallAbsorptivity=0.5  wallThermalK=1.4 % Parameterized on : 13-Jun-2026 10:47:25 W/(K*m)  winLength=1 m  winHeight=0.5 m  winThickness=0.007 m  winMaterialDen=2500 kg/m^3  winMaterialCp=787 J/(K*kg)  winAbsorptivity=0.35  winThermalK=1 W/(K*m)  winTransmissivity=0.45  ventLength=0.1 m  ventHeight=0.1 m  extToWallHTC=30 % Parameterized on : 13-Jun-2026 10:47:25 W/(K*m^2)  intToRoomHTC=30 % Parameterized on : 13-Jun-2026 10:47:25 W/(K*m^2)  iniT=300 % Parameterized on : 13-Jun-2026 10:47:25 K
  W_A4R1_A4R2 : WallSelector_lib/Wall Selector  optWall=wallModelOption.wallOnly  wallLength=0.00046 % Parameterized on : 13-Jun-2026 10:47:14 m  wallHeight=3.048 % Parameterized on : 13-Jun-2026 10:47:14 m  wallThickness=0.04 % Parameterized on : 13-Jun-2026 10:47:14 m  wallMaterialDen=650 % Parameterized on : 13-Jun-2026 10:47:25 kg/m^3  wallMaterialCp=1100 % Parameterized on : 13-Jun-2026 10:47:25 J/(K*kg)  wallAbsorptivity=0.5  wallThermalK=1.4 % Parameterized on : 13-Jun-2026 10:47:25 W/(K*m)  winLength=1 m  winHeight=0.5 m  winThickness=0.007 m  winMaterialDen=2500 kg/m^3  winMaterialCp=787 J/(K*kg)  winAbsorptivity=0.35  winThermalK=1 W/(K*m)  winTransmissivity=0.45  ventLength=0.1 m  ventHeight=0.1 m  extToWallHTC=30 % Parameterized on : 13-Jun-2026 10:47:25 W/(K*m^2)  intToRoomHTC=30 % Parameterized on : 13-Jun-2026 10:47:25 W/(K*m^2)  iniT=300 % Parameterized on : 13-Jun-2026 10:47:25 K
  W_A4R1_A4R3 : WallSelector_lib/Wall Selector  optWall=wallModelOption.wallOnly  wallLength=3.9624 % Parameterized on : 13-Jun-2026 10:47:14 m  wallHeight=3.048 % Parameterized on : 13-Jun-2026 10:47:14 m  wallThickness=0.04 % Parameterized on : 13-Jun-2026 10:47:14 m  wallMaterialDen=650 % Parameterized on : 13-Jun-2026 10:47:25 kg/m^3  wallMaterialCp=1100 % Parameterized on : 13-Jun-2026 10:47:25 J/(K*kg)  wallAbsorptivity=0.5  wallThermalK=1.4 % Parameterized on : 13-Jun-2026 10:47:25 W/(K*m)  winLength=1 m  winHeight=0.5 m  winThickness=0.007 m  winMaterialDen=2500 kg/m^3  winMaterialCp=787 J/(K*kg)  winAbsorptivity=0.35  winThermalK=1 W/(K*m)  winTransmissivity=0.45  ventLength=0.1 m  ventHeight=0.1 m  extToWallHTC=30 % Parameterized on : 13-Jun-2026 10:47:25 W/(K*m^2)  intToRoomHTC=30 % Parameterized on : 13-Jun-2026 10:47:25 W/(K*m^2)  iniT=300 % Parameterized on : 13-Jun-2026 10:47:25 K
  W_A4R1_A4R4 : WallSelector_lib/Wall Selector  optWall=wallModelOption.wallOnly  wallLength=3.6576 % Parameterized on : 13-Jun-2026 10:47:14 m  wallHeight=3.048 % Parameterized on : 13-Jun-2026 10:47:14 m  wallThickness=0.04 % Parameterized on : 13-Jun-2026 10:47:14 m  wallMaterialDen=650 % Parameterized on : 13-Jun-2026 10:47:25 kg/m^3  wallMaterialCp=1100 % Parameterized on : 13-Jun-2026 10:47:25 J/(K*kg)  wallAbsorptivity=0.5  wallThermalK=1.4 % Parameterized on : 13-Jun-2026 10:47:25 W/(K*m)  winLength=1 m  winHeight=0.5 m  winThickness=0.007 m  winMaterialDen=2500 kg/m^3  winMaterialCp=787 J/(K*kg)  winAbsorptivity=0.35  winThermalK=1 W/(K*m)  winTransmissivity=0.45  ventLength=0.1 m  ventHeight=0.1 m  extToWallHTC=30 % Parameterized on : 13-Jun-2026 10:47:25 W/(K*m^2)  intToRoomHTC=30 % Parameterized on : 13-Jun-2026 10:47:25 W/(K*m^2)  iniT=300 % Parameterized on : 13-Jun-2026 10:47:25 K
  W_A4R1_A4R5 : WallSelector_lib/Wall Selector  optWall=wallModelOption.wallOnly  wallLength=0.6096 % Parameterized on : 13-Jun-2026 10:47:14 m  wallHeight=3.048 % Parameterized on : 13-Jun-2026 10:47:14 m  wallThickness=0.04 % Parameterized on : 13-Jun-2026 10:47:14 m  wallMaterialDen=650 % Parameterized on : 13-Jun-2026 10:47:25 kg/m^3  wallMaterialCp=1100 % Parameterized on : 13-Jun-2026 10:47:25 J/(K*kg)  wallAbsorptivity=0.5  wallThermalK=1.4 % Parameterized on : 13-Jun-2026 10:47:25 W/(K*m)  winLength=1 m  winHeight=0.5 m  winThickness=0.007 m  winMaterialDen=2500 kg/m^3  winMaterialCp=787 J/(K*kg)  winAbsorptivity=0.35  winThermalK=1 W/(K*m)  winTransmissivity=0.45  ventLength=0.1 m  ventHeight=0.1 m  extToWallHTC=30 % Parameterized on : 13-Jun-2026 10:47:25 W/(K*m^2)  intToRoomHTC=30 % Parameterized on : 13-Jun-2026 10:47:25 W/(K*m^2)  iniT=300 % Parameterized on : 13-Jun-2026 10:47:25 K
  W_A4R1_A4R6 : WallSelector_lib/Wall Selector  optWall=wallModelOption.wallOnly  wallLength=0.9144 % Parameterized on : 13-Jun-2026 10:47:14 m  wallHeight=3.048 % Parameterized on : 13-Jun-2026 10:47:14 m  wallThickness=0.04 % Parameterized on : 13-Jun-2026 10:47:14 m  wallMaterialDen=650 % Parameterized on : 13-Jun-2026 10:47:25 kg/m^3  wallMaterialCp=1100 % Parameterized on : 13-Jun-2026 10:47:25 J/(K*kg)  wallAbsorptivity=0.5  wallThermalK=1.4 % Parameterized on : 13-Jun-2026 10:47:25 W/(K*m)  winLength=1 m  winHeight=0.5 m  winThickness=0.007 m  winMaterialDen=2500 kg/m^3  winMaterialCp=787 J/(K*kg)  winAbsorptivity=0.35  winThermalK=1 W/(K*m)  winTransmissivity=0.45  ventLength=0.1 m  ventHeight=0.1 m  extToWallHTC=30 % Parameterized on : 13-Jun-2026 10:47:25 W/(K*m^2)  intToRoomHTC=30 % Parameterized on : 13-Jun-2026 10:47:25 W/(K*m^2)  iniT=300 % Parameterized on : 13-Jun-2026 10:47:25 K
  W_A4R1_A4R7 : WallSelector_lib/Wall Selector  optWall=wallModelOption.wallOnly  wallLength=0.00046 % Parameterized on : 13-Jun-2026 10:47:14 m  wallHeight=3.048 % Parameterized on : 13-Jun-2026 10:47:14 m  wallThickness=0.04 % Parameterized on : 13-Jun-2026 10:47:14 m  wallMaterialDen=650 % Parameterized on : 13-Jun-2026 10:47:25 kg/m^3  wallMaterialCp=1100 % Parameterized on : 13-Jun-2026 10:47:25 J/(K*kg)  wallAbsorptivity=0.5  wallThermalK=1.4 % Parameterized on : 13-Jun-2026 10:47:25 W/(K*m)  winLength=1 m  winHeight=0.5 m  winThickness=0.007 m  winMaterialDen=2500 kg/m^3  winMaterialCp=787 J/(K*kg)  winAbsorptivity=0.35  winThermalK=1 W/(K*m)  winTransmissivity=0.45  ventLength=0.1 m  ventHeight=0.1 m  extToWallHTC=30 % Parameterized on : 13-Jun-2026 10:47:25 W/(K*m^2)  intToRoomHTC=30 % Parameterized on : 13-Jun-2026 10:47:25 W/(K*m^2)  iniT=300 % Parameterized on : 13-Jun-2026 10:47:25 K
  W_A4R2_A4R3 : WallSelector_lib/Wall Selector  optWall=wallModelOption.wallOnly  wallLength=0.00046 % Parameterized on : 13-Jun-2026 10:47:14 m  wallHeight=3.048 % Parameterized on : 13-Jun-2026 10:47:14 m  wallThickness=0.04 % Parameterized on : 13-Jun-2026 10:47:14 m  wallMaterialDen=650 % Parameterized on : 13-Jun-2026 10:47:25 kg/m^3  wallMaterialCp=1100 % Parameterized on : 13-Jun-2026 10:47:25 J/(K*kg)  wallAbsorptivity=0.5  wallThermalK=1.4 % Parameterized on : 13-Jun-2026 10:47:25 W/(K*m)  winLength=1 m  winHeight=0.5 m  winThickness=0.007 m  winMaterialDen=2500 kg/m^3  winMaterialCp=787 J/(K*kg)  winAbsorptivity=0.35  winThermalK=1 W/(K*m)  winTransmissivity=0.45  ventLength=0.1 m  ventHeight=0.1 m  extToWallHTC=30 % Parameterized on : 13-Jun-2026 10:47:25 W/(K*m^2)  intToRoomHTC=30 % Parameterized on : 13-Jun-2026 10:47:25 W/(K*m^2)  iniT=300 % Parameterized on : 13-Jun-2026 10:47:25 K
  W_A4R2_A4R4 : WallSelector_lib/Wall Selector  optWall=wallModelOption.wallOnly  wallLength=0.00046 % Parameterized on : 13-Jun-2026 10:47:14 m  wallHeight=3.048 % Parameterized on : 13-Jun-2026 10:47:14 m  wallThickness=0.04 % Parameterized on : 13-Jun-2026 10:47:14 m  wallMaterialDen=650 % Parameterized on : 13-Jun-2026 10:47:25 kg/m^3  wallMaterialCp=1100 % Parameterized on : 13-Jun-2026 10:47:25 J/(K*kg)  wallAbsorptivity=0.5  wallThermalK=1.4 % Parameterized on : 13-Jun-2026 10:47:25 W/(K*m)  winLength=1 m  winHeight=0.5 m  winThickness=0.007 m  winMaterialDen=2500 kg/m^3  winMaterialCp=787 J/(K*kg)  winAbsorptivity=0.35  winThermalK=1 W/(K*m)  winTransmissivity=0.45  ventLength=0.1 m  ventHeight=0.1 m  extToWallHTC=30 % Parameterized on : 13-Jun-2026 10:47:25 W/(K*m^2)  intToRoomHTC=30 % Parameterized on : 13-Jun-2026 10:47:25 W/(K*m^2)  iniT=300 % Parameterized on : 13-Jun-2026 10:47:25 K
  W_A4R3_A4R5 : WallSelector_lib/Wall Selector  optWall=wallModelOption.wallOnly  wallLength=0.0004 % Parameterized on : 13-Jun-2026 10:47:14 m  wallHeight=3.048 % Parameterized on : 13-Jun-2026 10:47:14 m  wallThickness=0.04 % Parameterized on : 13-Jun-2026 10:47:14 m  wallMaterialDen=650 % Parameterized on : 13-Jun-2026 10:47:25 kg/m^3  wallMaterialCp=1100 % Parameterized on : 13-Jun-2026 10:47:25 J/(K*kg)  wallAbsorptivity=0.5  wallThermalK=1.4 % Parameterized on : 13-Jun-2026 10:47:25 W/(K*m)  winLength=1 m  winHeight=0.5 m  winThickness=0.007 m  winMaterialDen=2500 kg/m^3  winMaterialCp=787 J/(K*kg)  winAbsorptivity=0.35  winThermalK=1 W/(K*m)  winTransmissivity=0.45  ventLength=0.1 m  ventHeight=0.1 m  extToWallHTC=30 % Parameterized on : 13-Jun-2026 10:47:25 W/(K*m^2)  intToRoomHTC=30 % Parameterized on : 13-Jun-2026 10:47:25 W/(K*m^2)  iniT=300 % Parameterized on : 13-Jun-2026 10:47:25 K
  W_A4R4_A4R6 : WallSelector_lib/Wall Selector  optWall=wallModelOption.wallOnly  wallLength=0.00037 % Parameterized on : 13-Jun-2026 10:47:14 m  wallHeight=3.048 % Parameterized on : 13-Jun-2026 10:47:14 m  wallThickness=0.04 % Parameterized on : 13-Jun-2026 10:47:14 m  wallMaterialDen=650 % Parameterized on : 13-Jun-2026 10:47:25 kg/m^3  wallMaterialCp=1100 % Parameterized on : 13-Jun-2026 10:47:25 J/(K*kg)  wallAbsorptivity=0.5  wallThermalK=1.4 % Parameterized on : 13-Jun-2026 10:47:25 W/(K*m)  winLength=1 m  winHeight=0.5 m  winThickness=0.007 m  winMaterialDen=2500 kg/m^3  winMaterialCp=787 J/(K*kg)  winAbsorptivity=0.35  winThermalK=1 W/(K*m)  winTransmissivity=0.45  ventLength=0.1 m  ventHeight=0.1 m  extToWallHTC=30 % Parameterized on : 13-Jun-2026 10:47:25 W/(K*m^2)  intToRoomHTC=30 % Parameterized on : 13-Jun-2026 10:47:25 W/(K*m^2)  iniT=300 % Parameterized on : 13-Jun-2026 10:47:25 K
  W_A4R5_A4R7 : WallSelector_lib/Wall Selector  optWall=wallModelOption.wallOnly  wallLength=1.524 % Parameterized on : 13-Jun-2026 10:47:14 m  wallHeight=3.048 % Parameterized on : 13-Jun-2026 10:47:14 m  wallThickness=0.04 % Parameterized on : 13-Jun-2026 10:47:14 m  wallMaterialDen=650 % Parameterized on : 13-Jun-2026 10:47:25 kg/m^3  wallMaterialCp=1100 % Parameterized on : 13-Jun-2026 10:47:25 J/(K*kg)  wallAbsorptivity=0.5  wallThermalK=1.4 % Parameterized on : 13-Jun-2026 10:47:25 W/(K*m)  winLength=1 m  winHeight=0.5 m  winThickness=0.007 m  winMaterialDen=2500 kg/m^3  winMaterialCp=787 J/(K*kg)  winAbsorptivity=0.35  winThermalK=1 W/(K*m)  winTransmissivity=0.45  ventLength=0.1 m  ventHeight=0.1 m  extToWallHTC=30 % Parameterized on : 13-Jun-2026 10:47:25 W/(K*m^2)  intToRoomHTC=30 % Parameterized on : 13-Jun-2026 10:47:25 W/(K*m^2)  iniT=300 % Parameterized on : 13-Jun-2026 10:47:25 K
  W_A4R6_A4R7 : WallSelector_lib/Wall Selector  optWall=wallModelOption.wallOnly  wallLength=1.524 % Parameterized on : 13-Jun-2026 10:47:14 m  wallHeight=3.048 % Parameterized on : 13-Jun-2026 10:47:14 m  wallThickness=0.04 % Parameterized on : 13-Jun-2026 10:47:14 m  wallMaterialDen=650 % Parameterized on : 13-Jun-2026 10:47:25 kg/m^3  wallMaterialCp=1100 % Parameterized on : 13-Jun-2026 10:47:25 J/(K*kg)  wallAbsorptivity=0.5  wallThermalK=1.4 % Parameterized on : 13-Jun-2026 10:47:25 W/(K*m)  winLength=1 m  winHeight=0.5 m  winThickness=0.007 m  winMaterialDen=2500 kg/m^3  winMaterialCp=787 J/(K*kg)  winAbsorptivity=0.35  winThermalK=1 W/(K*m)  winTransmissivity=0.45  ventLength=0.1 m  ventHeight=0.1 m  extToWallHTC=30 % Parameterized on : 13-Jun-2026 10:47:25 W/(K*m^2)  intToRoomHTC=30 % Parameterized on : 13-Jun-2026 10:47:25 W/(K*m^2)  iniT=300 % Parameterized on : 13-Jun-2026 10:47:25 K
  roomT : Subsystem
  Amb : PMIOPort  Side=Left
  Solar : PMIOPort  Port=2  Side=Left
  S : PMIOPort  Port=3  Side=Left
  Top : PMIOPort  Port=4  Side=Left
  T : PMIOPort  Port=5  Side=Right
  Bottom : PMIOPort  Port=6  Side=Right
  connections:
  Room_A1R1_LivingRoom_A/RConn1 -- W_A1R1_A1R2/RConn1
  W_A1R1_A1R2/LConn1 -- Room_A1R2_Bedroom_A/LConn2 -- W_A1R2_A1R3/RConn1 -- W_A1R2_A1R4/RConn1 -- ExtWall (A1R2W1)/RConn1
  W_A1R1_A1R3/RConn1 -- Room_A1R1_LivingRoom_A/LConn3 -- W_A1R1_A1R5/RConn1
  Room_A1R3_Kitchen_A/RConn3 -- W_A1R1_A1R3/LConn1
  W_A1R1_A1R4/RConn1 -- Room_A1R1_LivingRoom_A/RConn3 -- W_A1R1_A1R6/RConn1
  Room_A1R4_Bathroom_A/LConn3 -- W_A1R1_A1R4/LConn1
  W_A1R1_A1R5/LConn1 -- Room_A1R5_FireExit_A/RConn3 -- W_A1R5_A1R7/RConn1
  W_A1R1_A1R6/LConn1 -- Room_A1R6_Lobby1_A/LConn3 -- W_A1R6_A1R7/RConn1
  Room_A1R1_LivingRoom_A/LConn2 -- W_A1R1_A1R7/RConn1
  Room_A1R7_Lobby2_A/RConn1 -- W_A1R1_A1R7/LConn1
  W_A1R2_A1R3/LConn1 -- Room_A1R3_Kitchen_A/RConn1 -- ExtWall (A1R3W3)/RConn1
  W_A1R2_A1R4/LConn1 -- Room_A1R4_Bathroom_A/RConn1 -- ExtWall (A1R4W3)/RConn1
  W_A1R3_A1R5/RConn1 -- Room_A1R3_Kitchen_A/LConn2 -- ExtWall (A1R3W1)/RConn1
  Room_A1R5_FireExit_A/RConn1 -- W_A1R3_A1R5/LConn1
  Room_A1R4_Bathroom_A/LConn2 -- W_A1R4_A1R6/RConn1
  Room_A1R6_Lobby1_A/RConn1 -- W_A1R4_A1R6/LConn1
  Room_A1R7_Lobby2_A/LConn3 -- W_A1R5_A1R7/LConn1
  Room_A1R7_Lobby2_A/RConn3 -- W_A1R6_A1R7/LConn1
  Room_A2R1_LivingRoom_B/LConn2 -- W_A2R1_A2R2/RConn1
  W_A2R1_A2R2/LConn1 -- Room_A2R2_Bedroom_B/RConn1 -- W_A2R2_A2R3/RConn1 -- W_A2R2_A2R4/RConn1 -- ExtWall (A2R2W3)/RConn1
  W_A2R1_A2R3/RConn1 -- Room_A2R1_LivingRoom_B/LConn3 -- W_A2R1_A2R5/RConn1
  W_A2R1_A2R3/LConn1 -- Room_A2R3_Kitchen_B/RConn3 -- ExtWall (A2R3W2)/RConn1
  W_A2R1_A2R4/RConn1 -- Room_A2R1_LivingRoom_B/RConn3 -- W_A2R1_A2R6/RConn1
  Room_A2R4_Bathroom_B/LConn3 -- W_A2R1_A2R4/LConn1
  W_A2R1_A2R5/LConn1 -- Room_A2R5_FireExit_B/RConn3 -- W_A2R5_A2R7/RConn1 -- ExtWall (A2R5W2)/RConn1
  W_A2R1_A2R6/LConn1 -- Room_A2R6_Lobby1_B/LConn3 -- W_A2R6_A2R7/RConn1
  Room_A2R1_LivingRoom_B/RConn1 -- W_A2R1_A2R7/RConn1
  Room_A2R7_Lobby2_B/LConn2 -- W_A2R1_A2R7/LConn1
  W_A2R2_A2R3/LConn1 -- Room_A2R3_Kitchen_B/LConn2 -- ExtWall (A2R3W1)/RConn1
  Room_A2R4_Bathroom_B/LConn2 -- W_A2R2_A2R4/LConn1
  W_A2R3_A2R5/RConn1 -- Room_A2R3_Kitchen_B/RConn1 -- ExtWall (A2R3W3)/RConn1
  Room_A2R5_FireExit_B/LConn2 -- W_A2R3_A2R5/LConn1
  W_A2R4_A2R6/RConn1 -- Room_A2R4_Bathroom_B/RConn1 -- ExtWall (A2R4W3)/RConn1
  Room_A2R6_Lobby1_B/LConn2 -- W_A2R4_A2R6/LConn1
  Room_A2R7_Lobby2_B/LConn3 -- W_A2R5_A2R7/LConn1
  Room_A2R7_Lobby2_B/RConn3 -- W_A2R6_A2R7/LConn1
  Room_A3R1_LivingRoom_C/RConn1 -- W_A3R1_A3R2/RConn1
  W_A3R1_A3R2/LConn1 -- Room_A3R2_Bedroom_C/LConn2 -- W_A3R2_A3R3/RConn1 -- W_A3R2_A3R4/RConn1 -- ExtWall (A3R2W1)/RConn1
  W_A3R1_A3R3/RConn1 -- Room_A3R1_LivingRoom_C/RConn3 -- W_A3R1_A3R5/RConn1
  Room_A3R3_Kitchen_C/LConn3 -- W_A3R1_A3R3/LConn1
  W_A3R1_A3R4/RConn1 -- Room_A3R1_LivingRoom_C/LConn3 -- W_A3R1_A3R6/RConn1
  Room_A3R4_Bathroom_C/RConn3 -- W_A3R1_A3R4/LConn1
  W_A3R1_A3R5/LConn1 -- Room_A3R5_FireExit_C/LConn3 -- W_A3R5_A3R7/RConn1
  W_A3R1_A3R6/LConn1 -- Room_A3R6_Lobby1_C/RConn3 -- W_A3R6_A3R7/RConn1
  Room_A3R1_LivingRoom_C/LConn2 -- W_A3R1_A3R7/RConn1
  Room_A3R7_Lobby2_C/RConn1 -- W_A3R1_A3R7/LConn1
  W_A3R2_A3R3/LConn1 -- Room_A3R3_Kitchen_C/RConn1 -- ExtWall (A3R3W3)/RConn1
  W_A3R2_A3R4/LConn1 -- Room_A3R4_Bathroom_C/RConn1 -- ExtWall (A3R4W3)/RConn1
  W_A3R3_A3R5/RConn1 -- Room_A3R3_Kitchen_C/LConn2 -- ExtWall (A3R3W1)/RConn1
  Room_A3R5_FireExit_C/RConn1 -- W_A3R3_A3R5/LConn1
  Room_A3R4_Bathroom_C/LConn2 -- W_A3R4_A3R6/RConn1
  Room_A3R6_Lobby1_C/RConn1 -- W_A3R4_A3R6/LConn1
  Room_A3R7_Lobby2_C/RConn3 -- W_A3R5_A3R7/LConn1
  Room_A3R7_Lobby2_C/LConn3 -- W_A3R6_A3R7/LConn1
  Room_A4R1_LivingRoom_D/LConn2 -- W_A4R1_A4R2/RConn1
  W_A4R1_A4R2/LConn1 -- Room_A4R2_Bedroom_D/RConn1 -- W_A4R2_A4R3/RConn1 -- W_A4R2_A4R4/RConn1 -- ExtWall (A4R2W3)/RConn1
  W_A4R1_A4R3/RConn1 -- Room_A4R1_LivingRoom_D/RConn3 -- W_A4R1_A4R5/RConn1
  W_A4R1_A4R3/LConn1 -- Room_A4R3_Kitchen_D/LConn3 -- ExtWall (A4R3W4)/RConn1
  W_A4R1_A4R4/RConn1 -- Room_A4R1_LivingRoom_D/LConn3 -- W_A4R1_A4R6/RConn1
  Room_A4R4_Bathroom_D/RConn3 -- W_A4R1_A4R4/LConn1
  W_A4R1_A4R5/LConn1 -- Room_A4R5_FireExit_D/LConn3 -- W_A4R5_A4R7/RConn1 -- ExtWall (A4R5W4)/RConn1
  W_A4R1_A4R6/LConn1 -- Room_A4R6_Lobby1_D/RConn3 -- W_A4R6_A4R7/RConn1
  Room_A4R1_LivingRoom_D/RConn1 -- W_A4R1_A4R7/RConn1
  Room_A4R7_Lobby2_D/LConn2 -- W_A4R1_A4R7/LConn1
  W_A4R2_A4R3/LConn1 -- Room_A4R3_Kitchen_D/LConn2 -- ExtWall (A4R3W1)/RConn1
  Room_A4R4_Bathroom_D/LConn2 -- W_A4R2_A4R4/LConn1
  W_A4R3_A4R5/RConn1 -- Room_A4R3_Kitchen_D/RConn1 -- ExtWall (A4R3W3)/RConn1
  Room_A4R5_FireExit_D/LConn2 -- W_A4R3_A4R5/LConn1
  W_A4R4_A4R6/RConn1 -- Room_A4R4_Bathroom_D/RConn1 -- ExtWall (A4R4W3)/RConn1
  Room_A4R6_Lobby1_D/LConn2 -- W_A4R4_A4R6/LConn1
  Room_A4R7_Lobby2_D/RConn3 -- W_A4R5_A4R7/LConn1
  Room_A4R7_Lobby2_D/LConn3 -- W_A4R6_A4R7/LConn1
  ExtWall (A1R2W1)/LConn2 -- Amb1/LConn1
  Room_A1R2_Bedroom_A/RConn1 -- ExtWall (A1R2W3)/RConn1
  ExtWall (A1R2W3)/LConn2 -- Amb2/LConn1
  Room_A1R2_Bedroom_A/LConn3 -- ExtWall (A1R2W4)/RConn1
  ExtWall (A1R2W4)/LConn2 -- Amb3/LConn1
  ExtWall (A1R3W1)/LConn2 -- Amb4/LConn1
  ExtWall (A1R3W3)/LConn2 -- Amb5/LConn1
  Room_A1R3_Kitchen_A/LConn3 -- ExtWall (A1R3W4)/RConn1
  ExtWall (A1R3W4)/LConn2 -- Amb6/LConn1
  ExtWall (A1R4W3)/LConn2 -- Amb7/LConn1
  Room_A1R5_FireExit_A/LConn3 -- ExtWall (A1R5W4)/RConn1
  ExtWall (A1R5W4)/LConn2 -- Amb8/LConn1
  Room_A2R2_Bedroom_B/LConn2 -- ExtWall (A2R2W1)/RConn1
  ExtWall (A2R2W1)/LConn2 -- Amb9/LConn1
  Room_A2R2_Bedroom_B/RConn3 -- ExtWall (A2R2W2)/RConn1
  ExtWall (A2R2W2)/LConn2 -- Amb10/LConn1
  ExtWall (A2R2W3)/LConn2 -- Amb11/LConn1
  ExtWall (A2R3W1)/LConn2 -- Amb12/LConn1
  ExtWall (A2R3W2)/LConn2 -- Amb13/LConn1
  ExtWall (A2R3W3)/LConn2 -- Amb14/LConn1
  ExtWall (A2R4W3)/LConn2 -- Amb15/LConn1
  ExtWall (A2R5W2)/LConn2 -- Amb16/LConn1
  ExtWall (A3R2W1)/LConn2 -- Amb17/LConn1
  Room_A3R2_Bedroom_C/RConn3 -- ExtWall (A3R2W2)/RConn1
  ExtWall (A3R2W2)/LConn2 -- Amb18/LConn1
  Room_A3R2_Bedroom_C/RConn1 -- ExtWall (A3R2W3)/RConn1
  ExtWall (A3R2W3)/LConn2 -- Amb19/LConn1
  ExtWall (A3R3W1)/LConn2 -- Amb20/LConn1
  Room_A3R3_Kitchen_C/RConn3 -- ExtWall (A3R3W2)/RConn1
  ExtWall (A3R3W2)/LConn2 -- Amb21/LConn1
  ExtWall (A3R3W3)/LConn2 -- Amb22/LConn1
  ExtWall (A3R4W3)/LConn2 -- Amb23/LConn1
  Room_A3R5_FireExit_C/RConn3 -- ExtWall (A3R5W2)/RConn1
  ExtWall (A3R5W2)/LConn2 -- Amb24/LConn1
  Room_A4R2_Bedroom_D/LConn2 -- ExtWall (A4R2W1)/RConn1
  ExtWall (A4R2W1)/LConn2 -- Amb25/LConn1
  ExtWall (A4R2W3)/LConn2 -- Amb26/LConn1
  Room_A4R2_Bedroom_D/LConn3 -- ExtWall (A4R2W4)/RConn1
  ExtWall (A4R2W4)/LConn2 -- Amb27/LConn1
  ExtWall (A4R3W1)/LConn2 -- Amb28/LConn1
  ExtWall (A4R3W3)/LConn2 -- Amb29/LConn1
  ExtWall (A4R3W4)/LConn2 -- Amb30/LConn1
  ExtWall (A4R4W3)/LConn2 -- Amb31/LConn1
  ExtWall (A4R5W4)/LConn2 -- Amb32/LConn1
  Amb/RConn1 -- AmbPort/LConn1
  ExtWall (A1R2W1)/LConn1 -- ExtWall (A1R2W3)/LConn1 -- ExtWall (A1R2W4)/LConn1 -- ExtWall (A1R3W1)/LConn1 -- ExtWall (A1R3W3)/LConn1 -- ExtWall (A1R3W4)/LConn1 -- ExtWall (A1R4W3)/LConn1 -- ExtWall (A1R5W4)/LConn1 -- ExtWall (A2R2W1)/LConn1 -- ExtWall (A2R2W2)/LConn1 -- ExtWall (A2R2W3)/LConn1 -- ExtWall (A2R3W1)/LConn1 -- ExtWall (A2R3W2)/LConn1 -- ExtWall (A2R3W3)/LConn1 -- ExtWall (A2R4W3)/LConn1 -- ExtWall (A2R5W2)/LConn1 -- ExtWall (A3R2W1)/LConn1 -- ExtWall (A3R2W2)/LConn1 -- ExtWall (A3R2W3)/LConn1 -- ExtWall (A3R3W1)/LConn1 -- ExtWall (A3R3W2)/LConn1 -- ExtWall (A3R3W3)/LConn1 -- ExtWall (A3R4W3)/LConn1 -- ExtWall (A3R5W2)/LConn1 -- ExtWall (A4R2W1)/LConn1 -- ExtWall (A4R2W3)/LConn1 -- ExtWall (A4R2W4)/LConn1 -- ExtWall (A4R3W1)/LConn1 -- ExtWall (A4R3W3)/LConn1 -- ExtWall (A4R3W4)/LConn1 -- ExtWall (A4R4W3)/LConn1 -- Solar/RConn1 -- ExtWall (A4R5W4)/LConn1
  roomT/LConn1 -- Room_A1R1_LivingRoom_A/RConn2
  roomT/LConn2 -- Room_A1R2_Bedroom_A/RConn2
  roomT/LConn3 -- Room_A1R3_Kitchen_A/RConn2
  roomT/LConn4 -- Room_A1R4_Bathroom_A/RConn2
  roomT/LConn5 -- Room_A1R5_FireExit_A/RConn2
  roomT/LConn6 -- Room_A1R6_Lobby1_A/RConn2
  roomT/LConn7 -- Room_A1R7_Lobby2_A/RConn2
  roomT/LConn8 -- Room_A2R1_LivingRoom_B/RConn2
  roomT/LConn9 -- Room_A2R2_Bedroom_B/RConn2
  roomT/LConn10 -- Room_A2R3_Kitchen_B/RConn2
  roomT/LConn11 -- Room_A2R4_Bathroom_B/RConn2
  roomT/LConn12 -- Room_A2R5_FireExit_B/RConn2
  roomT/LConn13 -- Room_A2R6_Lobby1_B/RConn2
  roomT/LConn14 -- Room_A2R7_Lobby2_B/RConn2
  roomT/LConn15 -- Room_A3R1_LivingRoom_C/RConn2
  roomT/LConn16 -- Room_A3R2_Bedroom_C/RConn2
  roomT/LConn17 -- Room_A3R3_Kitchen_C/RConn2
  roomT/LConn18 -- Room_A3R4_Bathroom_C/RConn2
  roomT/LConn19 -- Room_A3R5_FireExit_C/RConn2
  roomT/LConn20 -- Room_A3R6_Lobby1_C/RConn2
  roomT/LConn21 -- Room_A3R7_Lobby2_C/RConn2
  roomT/LConn22 -- Room_A4R1_LivingRoom_D/RConn2
  roomT/LConn23 -- Room_A4R2_Bedroom_D/RConn2
  roomT/LConn24 -- Room_A4R3_Kitchen_D/RConn2
  roomT/LConn25 -- Room_A4R4_Bathroom_D/RConn2
  roomT/LConn26 -- Room_A4R5_FireExit_D/RConn2
  roomT/LConn27 -- Room_A4R6_Lobby1_D/RConn2
  roomT/LConn28 -- Room_A4R7_Lobby2_D/RConn2
  roomT/RConn1 -- T/RConn1
  Room_A1R1_LivingRoom_A/LConn1 -- Room_A1R2_Bedroom_A/LConn1 -- Room_A1R3_Kitchen_A/LConn1 -- Room_A1R4_Bathroom_A/LConn1 -- Room_A1R5_FireExit_A/LConn1 -- Room_A1R6_Lobby1_A/LConn1 -- Room_A1R7_Lobby2_A/LConn1 -- Room_A2R1_LivingRoom_B/LConn1 -- Room_A2R2_Bedroom_B/LConn1 -- Room_A2R3_Kitchen_B/LConn1 -- Room_A2R4_Bathroom_B/LConn1 -- Room_A2R5_FireExit_B/LConn1 -- Room_A2R6_Lobby1_B/LConn1 -- Room_A2R7_Lobby2_B/LConn1 -- Room_A3R1_LivingRoom_C/LConn1 -- Room_A3R2_Bedroom_C/LConn1 -- Room_A3R3_Kitchen_C/LConn1 -- Room_A3R4_Bathroom_C/LConn1 -- Room_A3R5_FireExit_C/LConn1 -- Room_A3R6_Lobby1_C/LConn1 -- Room_A3R7_Lobby2_C/LConn1 -- Room_A4R1_LivingRoom_D/LConn1 -- Room_A4R2_Bedroom_D/LConn1 -- Room_A4R3_Kitchen_D/LConn1 -- Room_A4R4_Bathroom_D/LConn1 -- Room_A4R5_FireExit_D/LConn1 -- Room_A4R6_Lobby1_D/LConn1 -- S/RConn1 -- Room_A4R7_Lobby2_D/LConn1
  Top1/LConn1 -- ArrayTop/LConn1
  Top2/LConn1 -- ArrayTop/LConn2
  Top3/LConn1 -- ArrayTop/LConn3
  Top4/LConn1 -- ArrayTop/LConn4
  Top5/LConn1 -- ArrayTop/LConn5
  Top6/LConn1 -- ArrayTop/LConn6
  Top7/LConn1 -- ArrayTop/LConn7
  Top8/LConn1 -- ArrayTop/LConn8
  Top9/LConn1 -- ArrayTop/LConn9
  Top10/LConn1 -- ArrayTop/LConn10
  Top11/LConn1 -- ArrayTop/LConn11
  Top12/LConn1 -- ArrayTop/LConn12
  Top13/LConn1 -- ArrayTop/LConn13
  Top14/LConn1 -- ArrayTop/LConn14
  Top15/LConn1 -- ArrayTop/LConn15
  Top16/LConn1 -- ArrayTop/LConn16
  Top17/LConn1 -- ArrayTop/LConn17
  Top18/LConn1 -- ArrayTop/LConn18
  Top19/LConn1 -- ArrayTop/LConn19
  Top20/LConn1 -- ArrayTop/LConn20
  Top21/LConn1 -- ArrayTop/LConn21
  Top22/LConn1 -- ArrayTop/LConn22
  Top23/LConn1 -- ArrayTop/LConn23
  Top24/LConn1 -- ArrayTop/LConn24
  Top25/LConn1 -- ArrayTop/LConn25
  Top26/LConn1 -- ArrayTop/LConn26
  Top27/LConn1 -- ArrayTop/LConn27
  Top28/LConn1 -- ArrayTop/LConn28
  ArrayTop/RConn1 -- Top/RConn1
  Room_A1R1_LivingRoom_A/LConn4 -- Top1Lib/LConn1
  Room_A1R2_Bedroom_A/LConn4 -- Top2Lib/LConn1
  Room_A1R3_Kitchen_A/LConn4 -- Top3Lib/LConn1
  Room_A1R4_Bathroom_A/LConn4 -- Top4Lib/LConn1
  Room_A1R5_FireExit_A/LConn4 -- Top5Lib/LConn1
  Room_A1R6_Lobby1_A/LConn4 -- Top6Lib/LConn1
  Room_A1R7_Lobby2_A/LConn4 -- Top7Lib/LConn1
  Room_A2R1_LivingRoom_B/LConn4 -- Top8Lib/LConn1
  Room_A2R2_Bedroom_B/LConn4 -- Top9Lib/LConn1
  Room_A2R3_Kitchen_B/LConn4 -- Top10Lib/LConn1
  Room_A2R4_Bathroom_B/LConn4 -- Top11Lib/LConn1
  Room_A2R5_FireExit_B/LConn4 -- Top12Lib/LConn1
  Room_A2R6_Lobby1_B/LConn4 -- Top13Lib/LConn1
  Room_A2R7_Lobby2_B/LConn4 -- Top14Lib/LConn1
  Room_A3R1_LivingRoom_C/LConn4 -- Top15Lib/LConn1
  Room_A3R2_Bedroom_C/LConn4 -- Top16Lib/LConn1
  Room_A3R3_Kitchen_C/LConn4 -- Top17Lib/LConn1
  Room_A3R4_Bathroom_C/LConn4 -- Top18Lib/LConn1
  Room_A3R5_FireExit_C/LConn4 -- Top19Lib/LConn1
  Room_A3R6_Lobby1_C/LConn4 -- Top20Lib/LConn1
  Room_A3R7_Lobby2_C/LConn4 -- Top21Lib/LConn1
  Room_A4R1_LivingRoom_D/LConn4 -- Top22Lib/LConn1
  Room_A4R2_Bedroom_D/LConn4 -- Top23Lib/LConn1
  Room_A4R3_Kitchen_D/LConn4 -- Top24Lib/LConn1
  Room_A4R4_Bathroom_D/LConn4 -- Top25Lib/LConn1
  Room_A4R5_FireExit_D/LConn4 -- Top26Lib/LConn1
  Room_A4R6_Lobby1_D/LConn4 -- Top27Lib/LConn1
  Room_A4R7_Lobby2_D/LConn4 -- Top28Lib/LConn1
  Bottom1/LConn1 -- ArrayBottom/LConn1
  Bottom2/LConn1 -- ArrayBottom/LConn2
  Bottom3/LConn1 -- ArrayBottom/LConn3
  Bottom4/LConn1 -- ArrayBottom/LConn4
  Bottom5/LConn1 -- ArrayBottom/LConn5
  Bottom6/LConn1 -- ArrayBottom/LConn6
  Bottom7/LConn1 -- ArrayBottom/LConn7
  Bottom8/LConn1 -- ArrayBottom/LConn8
  Bottom9/LConn1 -- ArrayBottom/LConn9
  Bottom10/LConn1 -- ArrayBottom/LConn10
  Bottom11/LConn1 -- ArrayBottom/LConn11
  Bottom12/LConn1 -- ArrayBottom/LConn12
  Bottom13/LConn1 -- ArrayBottom/LConn13
  Bottom14/LConn1 -- ArrayBottom/LConn14
  Bottom15/LConn1 -- ArrayBottom/LConn15
  Bottom16/LConn1 -- ArrayBottom/LConn16
  Bottom17/LConn1 -- ArrayBottom/LConn17
  Bottom18/LConn1 -- ArrayBottom/LConn18
  Bottom19/LConn1 -- ArrayBottom/LConn19
  Bottom20/LConn1 -- ArrayBottom/LConn20
  Bottom21/LConn1 -- ArrayBottom/LConn21
  Bottom22/LConn1 -- ArrayBottom/LConn22
  Bottom23/LConn1 -- ArrayBottom/LConn23
  Bottom24/LConn1 -- ArrayBottom/LConn24
  Bottom25/LConn1 -- ArrayBottom/LConn25
  Bottom26/LConn1 -- ArrayBottom/LConn26
  Bottom27/LConn1 -- ArrayBottom/LConn27
  Bottom28/LConn1 -- ArrayBottom/LConn28
  ArrayBottom/RConn1 -- Bottom/RConn1
  Room_A1R1_LivingRoom_A/RConn4 -- Bottom1Lib/LConn1
  Room_A1R2_Bedroom_A/RConn4 -- Bottom2Lib/LConn1
  Room_A1R3_Kitchen_A/RConn4 -- Bottom3Lib/LConn1
  Room_A1R4_Bathroom_A/RConn4 -- Bottom4Lib/LConn1
  Room_A1R5_FireExit_A/RConn4 -- Bottom5Lib/LConn1
  Room_A1R6_Lobby1_A/RConn4 -- Bottom6Lib/LConn1
  Room_A1R7_Lobby2_A/RConn4 -- Bottom7Lib/LConn1
  Room_A2R1_LivingRoom_B/RConn4 -- Bottom8Lib/LConn1
  Room_A2R2_Bedroom_B/RConn4 -- Bottom9Lib/LConn1
  Room_A2R3_Kitchen_B/RConn4 -- Bottom10Lib/LConn1
  Room_A2R4_Bathroom_B/RConn4 -- Bottom11Lib/LConn1
  Room_A2R5_FireExit_B/RConn4 -- Bottom12Lib/LConn1
  Room_A2R6_Lobby1_B/RConn4 -- Bottom13Lib/LConn1
  Room_A2R7_Lobby2_B/RConn4 -- Bottom14Lib/LConn1
  Room_A3R1_LivingRoom_C/RConn4 -- Bottom15Lib/LConn1
  Room_A3R2_Bedroom_C/RConn4 -- Bottom16Lib/LConn1
  Room_A3R3_Kitchen_C/RConn4 -- Bottom17Lib/LConn1
  Room_A3R4_Bathroom_C/RConn4 -- Bottom18Lib/LConn1
  Room_A3R5_FireExit_C/RConn4 -- Bottom19Lib/LConn1
  Room_A3R6_Lobby1_C/RConn4 -- Bottom20Lib/LConn1
  Room_A3R7_Lobby2_C/RConn4 -- Bottom21Lib/LConn1
  Room_A4R1_LivingRoom_D/RConn4 -- Bottom22Lib/LConn1
  Room_A4R2_Bedroom_D/RConn4 -- Bottom23Lib/LConn1
  Room_A4R3_Kitchen_D/RConn4 -- Bottom24Lib/LConn1
  Room_A4R4_Bathroom_D/RConn4 -- Bottom25Lib/LConn1
  Room_A4R5_FireExit_D/RConn4 -- Bottom26Lib/LConn1
  Room_A4R6_Lobby1_D/RConn4 -- Bottom27Lib/LConn1
  Room_A4R7_Lobby2_D/RConn4 -- Bottom28Lib/LConn1
